simulink model "HRES_ORC_PEM"  (R2025b)
settings: Solver=ode23t  StartTime=0.0  StopTime=35000  MaxStep=1728  RelTol=1e-3
model workspace (MAT data in the model file):
  CND_L = 10
  CND_T0 = 333.15
  CND_d = 0.012
  CND_n = 20
  CND_p0 = 150000
  GAS_Tmax = 430
  GAS_dT = 20
  GAS_kb = 0.04
  GAS_ki = 0.002
  GAS_kp = 0.05
  GAS_min = 0.02
  GAS_total = 5
  GAS_u0 = 0.05
  HRS_L = 10
  HRS_LG = 1
  HRS_d = 0.012
  HRS_n = 6
  HRS_nG = 25
  HRS_p0 = 0.3
  HRS_x0 = 0.2
  NOZ_kb = 0.025
  NOZ_ki = 0.0005
  NOZ_kp = 0.02
  NOZ_min = 0.01
  NOZ_u0 = 0.1
  ORC_T3set = 400
  ORC_Taux = -2
  ORC_Taux0 = 0
  ORC_kb = 0.4
  ORC_ki = 2e-07
  ORC_kp = 5e-07
  ORC_mdot0 = 0.2
  ORC_mmax = 1
  ORC_mmin = 0.01
  ORC_pset_MPa = 1
  RCV_V = 0.2
  RCV_frac0 = 0.5
  RCV_p0 = 0.15
  RCV_tau = 0.1
  TRB_Tref = 400
  TRB_mdot = 0.6
  TRB_pr = 6
values from neighbouring files (symbols this model uses):
  R_h2 = 4.12    [run_simulation.m]
libraries: fl_lib x62, nesl_utility x56, SimscapeFluids_lib x9, slpidlib x4, ee_lib x2
(part 4 of 5)

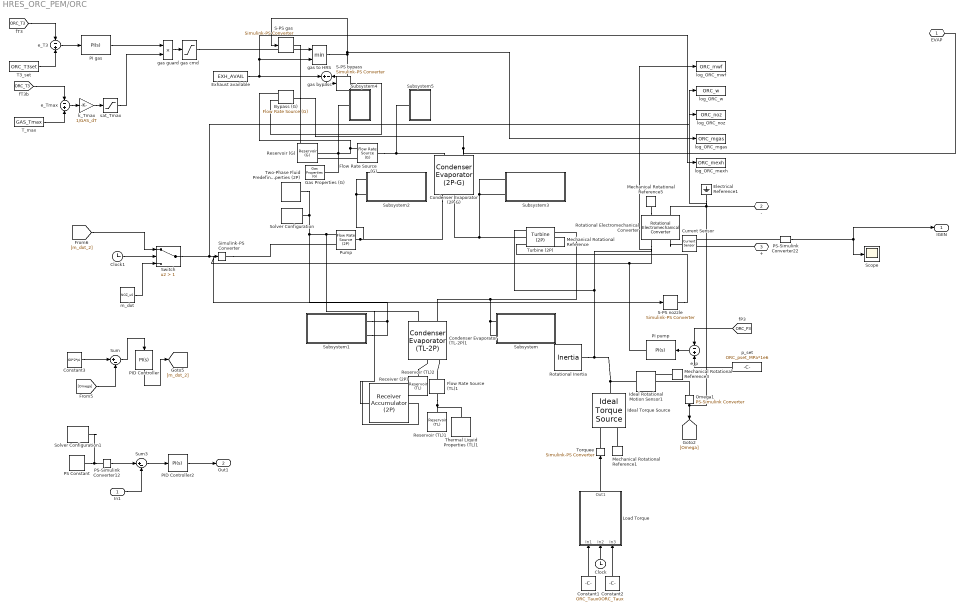
== system HRES_ORC_PEM/ORC ==
  In1 : Inport
  Bypass (G) : fl_lib/Gas/Sources/Flow Rate Source (G)  source_type=foundation.enum.constant_controlled.controlled  flow_type=foundation.enum.mass_volumetric_flow.mass  mass_flow=0 kg/s  volumetric_flow=0 m^3/s  volumetric_flow_conditions=foundation.enum.volumetric_flow_conditions.actual  p_std=0.101325 MPa  T_std=20 degC  power_spec=foundation.enum.power_spec.isentropic  area_A=0.01 m^2  area_B=0.01 m^2
      settings: InternalSimscapePortConfiguration="{\"Bottom\":[],\"Left\":[{\"id\":\"A\",\"label\":\"A\",\"type\":\"foundation.gas.gas\"},{\"id\":\"M\",\"label\":\"M\",\"type\":\"input\"}],\"Right\":[{\"id\":\"B\",\"label\":\"B\",\"type\":\"foundation.gas.gas\"}],\"Top\":[]}"
  Clock : Clock
  Clock1 : Clock
  Condenser Evaporator (2P-G) : SimscapeFluids_lib/Heat Exchangers/Two-Phase Fluid - Gas/Condenser Evaporator (2P-G)  flow_arrangement=fluids.heat_exchangers.enum.FlowArrangement2PG.Parallel  cross_flow_arrangement=fluids.heat_exchangers.enum.CrossFlowArrangement2PG.UnmixedUnmixed  R_wall=0 K/kW  wall_thermal_mass=false  mass_wall=1 kg  cp_wall=490 J/(K*kg)  area_A1=0.01 m^2  area_B1=0.01 m^2  area_A2=0.01 m^2  area_B2=0.01 m^2  tube_num_2P=HRS_n  tube_length_2P=HRS_L m  tube_cross_section_2P=fluids.heat_exchangers.enum.TubeCrossSection.Circular  tube_diameter_2P=HRS_d m  tube_width_2P=0.05 m  tube_height_2P=0.05 m  tube_inner_diameter_2P=0.05 m  tube_outer_diameter_2P=0.1 m  tube_flow_area_2P=0.002 m^2  tube_wetted_perimeter_2P=0.15 m  tube_heat_perimeter_2P=0.15 m  tube_pressure_loss_spec_2P=fluids.heat_exchangers.enum.TubePressureLossSpec2P.Haaland  tube_loss_coeff_2P=10  tube_local_pressure_loss_spec_2P=fluids.heat_exchangers.enum.LocalLossSpec.AggregateLength  tube_length_add_2P=0.1 m  tube_local_loss_coefficient_2P=0.1  tube_roughness_pressure_2P=15e-6 m  tube_Re_lam_pressure_2P=2000  tube_Re_tur_pressure_2P=4000  tube_shape_factor_generic_2P=64  tube_heat_coeff_spec_2P=fluids.heat_exchangers.enum.TubeHeatCoeffSpec2P.GneilinskiCavalliniZecchin  tube_colburn_coeff_liq_2P=[.023, .8, .33]  tube_colburn_coeff_mix_2P=[.05, .8, .33]  tube_colburn_coeff_vap_2P=[.023, .8, .33]  tube_roughness_heat_2P=15e-6 m  tube_Re_lam_heat_2P=2000  tube_Re_tur_heat_2P=4000  tube_Nu_lam_generic_2P=3.66  fouling_factor_2P=0.1 K*m^2/kW  fin_area_2P=0 m^2  fin_efficiency_2P=0.5  energy_spec_2P=foundation.enum.energy_spec.quality  p_init_2P=HRS_p0 MPa  T_init_2P=293.15 K  x_init_2P=HRS_x0  alpha_init_2P=0.5  h_init_2P=1500 kJ/kg  u_init_2P=1500 kJ/kg  flow_geometry_G=fluids.heat_exchangers.enum.FlowGeometryG.InsideTubes  tube_num_G=HRS_nG  tube_length_G=HRS_LG m  tube_cross_section_G=fluids.heat_exchangers.enum.TubeCrossSection.Circular  tube_diameter_G=0.05 m  tube_width_G=0.05 m  tube_height_G=0.05 m  tube_inner_diameter_G=0.05 m  tube_outer_diameter_G=0.1 m  tube_flow_area_G=0.002 m^2  tube_wetted_perimeter_G=0.15 m  tube_heat_perimeter_G=0.15 m  tube_pressure_loss_spec_G=fluids.heat_exchangers.enum.TubePressureLossSpec.Haaland  tube_loss_coeff_G=10  tube_local_pressure_loss_spec_G=fluids.heat_exchangers.enum.LocalLossSpec.AggregateLength  tube_length_add_G=0.1 m  tube_local_loss_coefficient_G=0.1  tube_roughness_pressure_G=15e-6 m  tube_Re_lam_pressure_G=2000  tube_Re_tur_pressure_G=4000  tube_shape_factor_generic_G=64  tube_heat_coeff_spec_G=fluids.heat_exchangers.enum.TubeHeatCoeffSpec.Gneilinski  tube_colburn_coeff_G=[.023, .8, .33]  tube_roughness_heat_G=15e-6 m  tube_Re_lam_heat_G=2000  tube_Re_tur_heat_G=4000  tube_Nu_lam_generic_G=3.66  bank_arrangement_G=fluids.heat_exchangers.enum.BankArrangement.Inline  bank_num_rows_G=5  bank_tubes_per_row_G=5  bank_width_G=1 m  bank_tube_diameter_G=0.05 m  bank_longitudinal_pitch_G=0.15 m  bank_transverse_pitch_G=0.15 m  bank_pressure_loss_spec_G=fluids.heat_exchangers.enum.BankPressureLossSpec.Martin  bank_euler_G=10  bank_heat_coeff_spec_G=fluids.heat_exchangers.enum.BankHeatCoeffSpec.Martin  bank_colburn_coeff_G=[.27, .63, .36]  generic_flow_area_G=0.01 m^2  generic_heat_area_G=2 m^2  generic_volume_G=0.05 m^3  generic_loss_coeff_G=10  generic_colburn_coeff_G=[.023, .8, .33]  fouling_factor_G=0.1 K*m^2/kW  fin_area_G=0 m^2  fin_efficiency_G=0.5  p_init_G=0.101325 MPa  T_init_G=453 K
      settings: InternalSimscapePortConfiguration="{\"Bottom\":[],\"Left\":[{\"id\":\"A1\",\"label\":\"A1\",\"type\":\"foundation.two_phase_fluid.two_phase_fluid\"},{\"id\":\"B1\",\"label\":\"B1\",\"type\":\"foundation.two_phase_fluid.two_phase_fluid\"}],\"Right\":[{\"id\":\"A2\",\"label\":\"A2\",\"type\":\"foundation.gas.gas\"},{\"id\":\"B2\",\"label\":\"B2\",\"type\":\"foundation.gas.gas\"}],\"Top\":[{\"id\":\"Z\",\"label\":\"Z\",\"type\":\"output\"}]}"
  Condenser Evaporator (TL-2P)1 : SimscapeFluids_lib/Heat Exchangers/Two-Phase Fluid - Thermal Liquid/Condenser Evaporator (TL-2P)  flow_arrangement=fluids.heat_exchangers.enum.FlowArrangementTL2P.Counter  cross_flow_arrangement=fluids.heat_exchangers.enum.CrossFlowArrangementTL2P.UnmixedUnmixed  R_wall=0 K/kW  wall_thermal_mass=false  mass_wall=1 kg  cp_wall=490 J/(K*kg)  area_A1=0.01 m^2  area_B1=0.01 m^2  area_A2=0.01 m^2  area_B2=0.01 m^2  flow_geometry_TL=fluids.heat_exchangers.enum.FlowGeometryTL.InsideTubes  tube_num_TL=40  tube_length_TL=1 m  tube_cross_section_TL=fluids.heat_exchangers.enum.TubeCrossSection.Circular  tube_diameter_TL=0.05 m  tube_width_TL=0.05 m  tube_height_TL=0.05 m  tube_inner_diameter_TL=0.05 m  tube_outer_diameter_TL=0.1 m  tube_flow_area_TL=0.002 m^2  tube_wetted_perimeter_TL=0.15 m  tube_heat_perimeter_TL=0.15 m  tube_pressure_loss_spec_TL=fluids.heat_exchangers.enum.TubePressureLossSpec.Haaland  tube_loss_coeff_TL=10  tube_local_pressure_loss_spec_TL=fluids.heat_exchangers.enum.LocalLossSpec.AggregateLength  tube_length_add_TL=0.1 m  tube_local_loss_coefficient_TL=0.1  tube_roughness_pressure_TL=15e-6 m  tube_Re_lam_pressure_TL=2000  tube_Re_tur_pressure_TL=4000  tube_shape_factor_generic_TL=64  tube_heat_coeff_spec_TL=fluids.heat_exchangers.enum.TubeHeatCoeffSpec.Gneilinski  tube_colburn_coeff_TL=[.023, .8, .33]  tube_roughness_heat_TL=15e-6 m  tube_Re_lam_heat_TL=2000  tube_Re_tur_heat_TL=4000  tube_Nu_lam_generic_TL=3.66  bank_arrangement_TL=fluids.heat_exchangers.enum.BankArrangement.Inline  bank_num_rows_TL=5  bank_tubes_per_row_TL=5  bank_width_TL=1 m  bank_tube_diameter_TL=0.05 m  bank_longitudinal_pitch_TL=0.15 m  bank_transverse_pitch_TL=0.15 m  bank_pressure_loss_spec_TL=fluids.heat_exchangers.enum.BankPressureLossSpec.Martin  bank_euler_TL=10  bank_heat_coeff_spec_TL=fluids.heat_exchangers.enum.BankHeatCoeffSpec.Martin  bank_colburn_coeff_TL=[.27, .63, .36]  generic_flow_area_TL=0.01 m^2  generic_heat_area_TL=2 m^2  generic_volume_TL=0.05 m^3  generic_loss_coeff_TL=10  generic_colburn_coeff_TL=[.023, .8, .33]  fouling_factor_TL=0.1 K*m^2/kW  fin_area_TL=0 m^2  fin_efficiency_TL=0.5  p_init_TL=99999 Pa  T_init_TL=275.15 K  tube_num_2P=CND_n  tube_length_2P=CND_L m  tube_cross_section_2P=fluids.heat_exchangers.enum.TubeCrossSection.Circular  tube_diameter_2P=CND_d m  tube_width_2P=0.05 m  tube_height_2P=0.05 m  tube_inner_diameter_2P=0.05 m  tube_outer_diameter_2P=0.1 m  tube_flow_area_2P=0.002 m^2  tube_wetted_perimeter_2P=0.15 m  tube_heat_perimeter_2P=0.15 m  tube_pressure_loss_spec_2P=fluids.heat_exchangers.enum.TubePressureLossSpec2P.Haaland  tube_loss_coeff_2P=10  tube_local_pressure_loss_spec_2P=fluids.heat_exchangers.enum.LocalLossSpec.AggregateLength  tube_length_add_2P=0.1 m  tube_local_loss_coefficient_2P=0.1  tube_roughness_pressure_2P=15e-6 m  tube_Re_lam_pressure_2P=2000  tube_Re_tur_pressure_2P=4000  tube_shape_factor_generic_2P=64  tube_heat_coeff_spec_2P=fluids.heat_exchangers.enum.TubeHeatCoeffSpec2P.GneilinskiCavalliniZecchin  tube_colburn_coeff_liq_2P=[.023, .8, .33]  tube_colburn_coeff_mix_2P=[.05, .8, .33]  tube_colburn_coeff_vap_2P=[.023, .8, .33]  tube_roughness_heat_2P=15e-6 m  tube_Re_lam_heat_2P=2000  tube_Re_tur_heat_2P=4000  tube_Nu_lam_generic_2P=3.66  fouling_factor_2P=0.1 K*m^2/kW  fin_area_2P=0 m^2  fin_efficiency_2P=0.5  energy_spec_2P=foundation.enum.energy_spec.temperature  p_init_2P=CND_p0 Pa  T_init_2P=CND_T0 K  x_init_2P=0.5  alpha_init_2P=0.5  h_init_2P=1500 kJ/kg  u_init_2P=1500 kJ/kg
      settings: InternalSimscapePortConfiguration="{\"Bottom\":[],\"Left\":[{\"id\":\"A1\",\"label\":\"A1\",\"type\":\"foundation.thermal_liquid.thermal_liquid\"},{\"id\":\"B1\",\"label\":\"B1\",\"type\":\"foundation.thermal_liquid.thermal_liquid\"}],\"Right\":[{\"id\":\"A2\",\"label\":\"A2\",\"type\":\"foundation.two_phase_fluid.two_phase_fluid\"},{\"id\":\"B2\",\"label\":\"B2\",\"type\":\"foundation.two_phase_fluid.two_phase_fluid\"}],\"Top\":[{\"id\":\"Z\",\"label\":\"Z\",\"type\":\"output\"}]}"
  Constant1 : Constant  Value=ORC_Taux0
  Constant2 : Constant  Value=ORC_Taux
  Constant3 : Constant  Value=60*2*pi
  Current Sensor : fl_lib/Electrical/Electrical Sensors/Current Sensor
  Electrical Reference1 : fl_lib/Electrical/Electrical Elements/Electrical Reference
  Exhaust available : FromWorkspace  VariableName=EXH_AVAIL  OutputAfterFinalValue=Holding final value
  Flow Rate Source (TL)1 : fl_lib/Thermal Liquid/Sources/Flow Rate Source (TL)  source_type=foundation.enum.constant_controlled.constant  flow_type=foundation.enum.mass_volumetric_flow.mass  mass_flow=15 kg/s  volumetric_flow=0 m^3/s  power_spec=foundation.enum.power_spec.isentropic  area=0.01 m^2
      settings: InternalSimscapePortConfiguration="{\"Bottom\":[],\"Left\":[{\"id\":\"A\",\"label\":\"A\",\"type\":\"foundation.thermal_liquid.thermal_liquid\"}],\"Right\":[{\"id\":\"B\",\"label\":\"B\",\"type\":\"foundation.thermal_liquid.thermal_liquid\"}],\"Top\":[]}"
  Flow Rate Source (G) : fl_lib/Gas/Sources/Flow Rate Source (G)  source_type=foundation.enum.constant_controlled.controlled  flow_type=foundation.enum.mass_volumetric_flow.mass  mass_flow=5 kg/s  volumetric_flow=0 m^3/s  volumetric_flow_conditions=foundation.enum.volumetric_flow_conditions.actual  p_std=0.101325 MPa  T_std=20 degC  power_spec=foundation.enum.power_spec.isentropic  area_A=0.01 m^2  area_B=0.01 m^2
      settings: InternalSimscapePortConfiguration="{\"Bottom\":[],\"Left\":[{\"id\":\"A\",\"label\":\"A\",\"type\":\"foundation.gas.gas\"},{\"id\":\"M\",\"label\":\"M\",\"type\":\"input\"}],\"Right\":[{\"id\":\"B\",\"label\":\"B\",\"type\":\"foundation.gas.gas\"}],\"Top\":[]}"
  Gas Properties (G) : fl_lib/Gas/Utilities/Gas Properties (G)  gas_spec=foundation.enum.gas_spec.perfect_gas  R=0.287 kJ/(K*kg)  Z=1  T_ref=293.15 K  h_ref=420 kJ/kg  cp_ref=1 kJ/(K*kg)  mu_ref=18 s*uPa  k_ref=26 mW/(K*m)  T_TLU1=[150 : 10 : 200, 250 : 50 : 1000, 1500, 2000]' K  h_TLU1=[275.264783730547; 285.377054177734; 295.474578903607; 305.560871069627; 315.638490783961; 325.709373787179; 376.008033649461; 426.297784741196; 476.678788323875; 527.253890684429; 578.12722735187; 629.395040865183; 681.137690131207; 733.415442873049; 786.267894376777; 839.715851152006; 893.764459999509; 948.406676876931; 1003.62653219711; 1059.40193232821; 1115.70691941005; 1172.51341226958; 1762.18512007361; 2377.14064127409] kJ/kg  cp_TLU1=[1.01211492398124; 1.01042105529234; 1.00914159006373; 1.00815898273273; 1.00739688341918; 1.00680484569075; 1.00554191216852; 1.00637389921747; 1.0092105862442; 1.01414404435034; 1.02111299587909; 1.02986878923959; 1.04003820504128; 1.05120320041448; 1.06296312852444; 1.07497111709439; 1.08694865668905; 1.0986858495625; 1.11003396604319; 1.12089493621399; 1.13121051694521; 1.14095251451866; 1.21001953144; 1.24628356718428] kJ/(K*kg)  mu_TLU1=[10.3766056544352; 10.9908682444892; 11.5932000841352; 12.1841060353213; 12.764067709023; 13.3335437107148; 16.038149065057; 18.5373404836509; 20.8671495114253; 23.0554226800681; 25.1239717991959; 27.0901379793485; 28.96790749834; 30.7687111230031; 32.5020036481173; 34.17569027566; 35.7964450415303; 37.3699520751368; 38.9010908824946; 40.3940804368247; 41.8525925389218; 43.279841956487; 56.3254722619962; 68.068290080945] s*uPa  k_TLU1=[14.1517155766309; 15.0474512994325; 15.9300520513026; 16.7998749295306; 17.6573089963228; 18.5027588910197; 22.5644026699512; 26.384465676638; 30.0032801168886; 33.4532006033488; 36.7600619429332; 39.9446251241844; 43.0237448740114; 46.0112537033799; 48.9186234516389; 51.7554617696538; 54.5298878921773; 57.2488200454925; 59.9181976996146; 62.5431553064749; 65.128159527924; 67.6771186900213; 91.7815514375552; 114.486299090693] mW/(K*m)  T_TLU2=[150 : 10 : 200, 250 : 50 : 1000, 1500, 2000]' K  p_TLU2=[0.001, 0.005, 0.01 : 0.01 : 0.1, 0.12, 0.15, 0.2, 0.5, 1, 2, 5, 10] MPa  rho_TLU2=[.0232262435294122, .116159536418799, .232389928446798, .465063671432694, .698022015548056, .931265751213184, 1.16479567270147, 1.39861257816015, 1.6327172696322, 1.86711055307826, 2.10179323839862, 2.33676613945539, 2.80758586416975, 3.5160126461103, 4.70263894299404, 11.983516436453, 24.7878864888476, 53.4753944012435, 188.202476404452, 488.088746553617; .0217743613495483, .108893511712, .217841319668304, .43590005028115, .654176644853253, .872671558133916, 1.09138524660849, 1.31031816850974, 1.52947078382145, 1.74884355428525, 1.96843694340691, 2.18825141646267, 2.62854548437173, 3.29065645015247, 4.39865940277095, 11.1676860192343, 22.9408518273177, 48.6188318442922, 151.41140977555, 397.086323615566; .0204933366521843, .102483510434793, .205009108095605, .410186693889784, .615533015460279, .821048331668635, 1.02673290215943, 1.23258698736378, 1.43861084849942, 1.64480474757224, 1.85116894737755, 2.05770371150129, 2.47128599100851, 3.09294527790581, 4.13249094693848, 10.4620818492884, 21.3797637857971, 44.7465382224065, 130.788260466556, 323.533424670971; .0193546817661166, .0967865758150396, .193606079729805, .38734394286521, .581213731637423, .775215588625983, .969349656759853, 1.16361607931376, 1.3580149999119, 1.55254656252557, 1.74721091147342, 1.94200819142115, 2.33200212471295, 2.91799364372034, 3.89732426996839, 9.84460606064557, 20.0372743829505, 41.551685035359, 116.744404785154, 273.404057887341; .0183359096145539, .0916899272240984, .183405807765996, .36691546510227, .55052904470126, .73424661940584, .918068262208759, 1.10199404625358, 1.28602404482977, 1.4701583313773, 1.65439697948324, 1.83874006288175, 2.20773983122517, 2.762024600182, 3.68793116346732, 9.2989642809239, 18.8669316601087, 38.8510263281099, 106.248040134752, 239.063674783047; .01741903255699, .0871033908068388, .174227353976232, .348537012803259, .52292900732162, .697403368434475, .871960127107058, 1.04659931436613, 1.22132096130094, 1.39612509905803, 1.57101175884641, 1.74598097193374, 2.09616718336943, 2.62206643530815, 3.50022045445381, 8.81280884432948, 17.8353318467781, 36.5262009931833, 97.9572133071041, 214.144269454883; .013935029468547, .069677797422131, .139362218300841, .278750918818379, .418166078341516, .557607673672086, .697075681624698, .836570079026588, .976090842717464, 1.11563794954935, 1.25521137638644, 1.39481110010495, 1.67408934575015, 2.09320336340731, 2.79224958681861, 7.00009934436889, 14.0635945083875, 28.3693859898697, 72.4958995959279, 148.061190553083; .0116124502542183, .0580629736195308, .116127751690325, .232262711724454, .348404861191252, .464554181197709, .580710652868886, .696874257347851, .813044975795622, .9292227893911, 1.04540767933102, 1.16159962682988, 1.3940046194509, 1.74266457145192, 2.32390314733333, 5.81485119489922, 11.6454651017326, 23.345179818482, 58.6036404676478, 116.933272564178; .0099534967844241, .0497674630503702, .0995348730218713, .199069527735142, .298603952162752, .39813813434232, .497672062326111, .597205724181, .696739107988446, .796272201844446, .89580499385952, .995337472158662, 1.19440144018133, 1.49299474329964, 1.99064239855983, 4.97624478331013, 9.95052507838832, 19.8877675359538, 49.5222664696343, 97.8281817865855; .00870929477376754, .0435461574066765, .0870915231079571, .174179875730153, .261265050544649, .348347040239765, .435425837514054, .522501435076285, .609573825645425, .696643001950612, .783708956731145, .870771682736456, 1.0448874194697, 1.30603662807179, 1.74121977223468, 4.35055112014231, 8.6923131825558, 17.3462098741118, 43.0204270425471, 84.5862815012905; .00774158811214905, .0387075144483394, .0774139632775453, .154823661826077, .232229091144957, .309630246740453, .387027124125729, .464419718820829, .541808026352667, .619192042255013, .696571762068483, .773947181340524, .92868510048419, 1.16075961421661, 1.54746386958083, 3.86538722275345, 7.71958432856407, 15.3924298760864, 38.0966874262009, 74.7409240194489; .00696742576213167, .0348366745541997, ...(+4677 chars)] kg/m^3  s_TLU2=[4.51795188269071, 4.05581817155212, 3.85666832168988, 3.65733557342939, 3.54058125651975, 3.45763599951791, 3.39321600973057, 3.34051347760226, 3.2958969095816, 3.25719862711102, 3.22302043260479, 3.19240764614444, 3.13933271586112, 3.07416650003008, 2.98972303348322, 2.71525667312277, 2.4961408855038, 2.25200576011077, 1.78471429674036, 1.29090458888978; 4.58264139768585, 4.12053027678858, 3.92140869957028, 3.72213261304626, 3.60543511368002, 3.52254683068083, 3.45818397201293, 3.40553872878098, 3.36097960809753, 3.32233893207258, 3.28821850379162, 3.25766364401107, 3.20470505116893, 3.13971456199421, 3.0555672742907, 2.78296953737326, 2.56736420779637, 2.33223141053168, 1.92951303779799, 1.47834112059833; 4.64340807746311, 4.18131468716962, 3.98221529565273, 3.7829836555054, 3.66633070274765, 3.58348706691023, 3.51916895627942, 3.46656856228366, 3.42205439236042, 3.38345876894588, 3.34938349545299, 3.31887389296688, 3.26600612355405, 3.20115264661303, 3.11723580728132, 2.84607806940339, 2.63311263769974, 2.40436393408814, 2.03542502560031, 1.64260706565665; 4.70070120514689, 4.23862199210925, 4.03954033696417, 3.84034421897669, 3.72372685440119, 3.64091887292993, 3.57663648301021, 3.52407187623307, 3.47959356019832, 3.44103385750504, 3.40699457172949, 3.37652102412054, 3.32372556659858, 3.25898106531012, 3.17524721731924, 2.90522439822934, 2.69430151549255, 2.47029333509785, 2.12268019468985, 1.77344207366055; 4.75489722787718, 4.29282953355363, 4.09376228675006, 3.89459501864723, 3.77800654829308, 3.6952275054615, 3.63097409868183, 3.57843851962613, 3.53398927597682, 3.49545869041481, 3.46144856659854, 3.43100422585914, 3.37826731713668, 3.31361097793741, 3.23002497599441, 2.96091365856363, 2.75160785927873, 2.5312406415135, 2.19841869007162, 1.87901583141216; 4.80631476306848, 4.34425655817633, 4.14520117995298, 3.94605767166668, 3.82949299137135, 3.74673776888186, 3.68250821276855, 3.6299965147449, 3.58557118253351, 3.54706453885701, 3.51307838741468, 3.48265804957869, 3.42996923841567, 3.36538527555295, 3.28192051690123, 3.0135531037355, 2.80555209686157, 2.58805540086205, 2.26610502263839, 1.96775904763196; 5.03005784939063, 4.56802897988245, 4.36901028390122, 4.16994018348893, 4.05344896894834, 3.97076727012748, 3.90661129562974, 3.85417323720152, 3.80982160259854, 3.77138871457567, 3.73747637686492, 3.70712991087092, 3.65458901785221, 3.59022736883767, 3.5071342997304, 3.24102784511277, 3.03691403727937, 2.82764560970477, 2.53381584725277, 2.28577338343632; 5.213071332015, 4.75105689184319, 4.55205623466113, 4.35302221894054, 4.23656709854542, 4.15392150331888, 4.08980164185938, 4.03739970590832, 3.99308420321641, 3.95468745653345, 3.92081126958634, 3.89050096377458, 3.83803241935538, 3.77377936374874, 3.69086747132005, 3.42585296452877, 3.22357730852106, 3.01804958620108, 2.73582153398541, 2.50683391368241; 5.36818677114197, 4.90618047542133, 4.70718999888292, 4.5081763447144, 4.391741586223, 4.30911635325018, 4.24501685439271, 4.19263528139031, 4.14834014199198, 4.10996375894582, 4.07610793597701, 4.04581799448331, 3.99339017971249, 3.92919822108258, 3.84638816350602, 3.58198482518679, 3.38072826636793, 3.17723930571407, 2.90109390657126, 2.68174878534546; 5.50312059773904, 5.04111933360368, 4.84213514624873, 4.64313406945348, 4.52671188701069, 4.444099228762, 4.38001230330443, 4.32764330237786, 4.28336073373153, 4.2449969201137, 4.21115366524977, 4.18087629053765, 4.12847360536087, 4.06431933120169, 3.98157205463241, 3.71754470888327, 3.51691216187067, 3.31466120289276, 3.04214220284213, 2.82845136827457; 5.62286980836317, 5.16087185851824, 4.96189181371153, 4.76289902096378, 4.64648512117041, 4.5638807441738, 4.49980209857165, 4.44744137610457, 4.40316708452248, 4.36481154657435, 4.33097656598627, 4.30070746415684, 4.24832132056873, 4.184191848361, 4.10148588060503, 3.83770566300567, 3.63748226836764, 3.43603958793625, 3.1658665252885, 2.9558053312017; 5.7308363809493, 5.26884072164272, 5.06986353974934, ...(+4595 chars)] kJ/(K*kg)  h_TLU2=[276.08088424589, 276.048494255671, 276.007989595737, 275.926922934925, 275.845779642901, 275.764559507019, 275.68326231383, 275.601887849085, 275.520435897725, 275.438906243879, 275.357298670861, 275.275612961165, 275.112006257597, 274.86600469197, 274.45440990197, 271.941510053176, 267.573991878308, 258.028969756929, 218.234362269026, 158.930370089034; 286.104280121225, 286.075386875978, 286.039258534729, 285.966962517021, 285.894613959392, 285.822212750054, 285.749758776967, 285.677251927836, 285.604692090115, 285.532079151003, 285.459412997448, 285.386693516142, 285.241094115775, 285.02229220976, 284.656540566853, 282.432853052032, 278.608576829258, 270.456137821523, 240.62825338508, 187.975341616082; 296.127712933609, 296.101741810155, 296.069269816893, 296.004298839236, 295.939291824284, 295.874248713054, 295.809169446516, 295.744053965591, 295.678902211156, 295.613714124043, 295.548489645037, 295.483228714877, 295.352597263841, 295.15637521962, 294.828601531559, 292.84221621424, 289.452931620771, 282.352183856267, 258.083267319111, 215.051052511419; 306.15128235, 306.127789707445, 306.098418400666, 306.03965742714, 305.980871947927, 305.922061932168, 305.863227349031, 305.804368167707, 305.745484357418, 305.686575887409, 305.627642726955, 305.568684845356, 305.450694796075, 305.273523547766, 304.977739633649, 303.189749788045, 300.157496456351, 293.885241012016, 273.341211471863, 237.921819553097; 316.175106263887, 316.153742662618, 316.127034494775, 316.073605930689, 316.02016104886, 315.966699833479, 315.913222268783, 315.859728339056, 315.806218028628, 315.752691321877, 315.69914820323, 315.64558865716, 315.538420220892, 315.377543975481, 315.109086307672, 313.489564435311, 310.756170955578, 305.156737704007, 287.344997830989, 257.435968836394; 326.199329972833, 326.179815330189, 326.155419682752, 326.106620570346, 326.057811027999, 326.008991047875, 325.960160622186, 325.911319743189, 325.862468403192, 325.813606594551, 325.764734309671, 325.715851541006, 325.61805452238, 325.471280180241, 325.226445621544, 323.751863790821, 321.272681065641, 316.232458831075, 300.538097964225, 274.729457520261; 376.334239729127, 376.321229547392, 376.304967312284, 376.272444481832, 376.239923836974, 376.207405376818, 376.174889100496, 376.142375007157, 376.109863095975, 376.077353366143, 376.044845816876, 376.012340447409, 375.94733624493, 375.849846271845, 375.687406489001, 374.713906995184, 373.095751316588, 369.876236784684, 360.387900683659, 345.656435942873; 426.525281394678, 426.516201936382, 426.50485367445, 426.482160685975, 426.459472409486, 426.436788842749, 426.414109983542, 426.391435829652, 426.36876637888, 426.346101629033, 426.323441577933, 426.30078622341, 426.255489595469, 426.18757982426, 426.074490520224, 425.398399641627, 424.280795394447, 422.079563123224, 415.746855514936, 406.194464895021; 476.840330742115, 476.833880716237, 476.825819267465, 476.80969998052, 476.793585505402, 476.777475839349, 476.761370979607, 476.745270923427, 476.729175668068, 476.713085210797, 476.696999548886, 476.680918679615, 476.648771308144, 476.600586128119, 476.520372988485, 476.041583484634, 475.252944483118, 473.709732112807, 469.339610018801, 462.897504479846; 527.36836576253, 527.363793291798, 527.358078674724, 527.346652677109, 527.335230992635, 527.323813618625, 527.312400552407, 527.300991791313, 527.289587332681, 527.278187173855, 527.26679131218, 527.255399745011, 527.232629483622, 527.198506234422, 527.141719692163, 526.803228763503, 526.247426409769, 525.16611881262, 522.148839900958, 517.815837109305; 578.206537117266, 578.203367844661, 578.199407091628, 578.191488376844, 578.183573381787, 578.175662104083, 578.16775454136, 578.159850691251, 578.151950551393, 578.144054119424, 578.136161392988, 578.128272369734, 578.112505423374, 578.088882719087, 578.049585297172, 577.815721490642, 577.433139940652, 576.694019389874, 574.669839072011, 571.873288825611; 629.447171720403, 629.445087134045, 629.442482115764, ...(+4600 chars)] kJ/kg  cp_TLU2=[1.00234082589656, 1.00272486727657, 1.00320557010184, 1.0041691525775, 1.00513564892549, 1.00610507294701, 1.00707743852905, 1.00805275964505, 1.00903105035552, 1.01001232480866, 1.01099659724104, 1.01198388197822, 1.01396754611819, 1.01696599794404, 1.02202562270308, 1.05412155485561, 1.1152747482059, 1.27776397304517, 2.72714600163742, 2.84169679152775; 1.00233987250094, 1.0026582461868, 1.00305665529268, 1.00385495020235, 1.00465521997313, 1.00545747174991, 1.00626171270995, 1.00706795006302, 1.00787619105157, 1.00868644295088, 1.00949871306922, 1.01031300874797, 1.01194770631902, 1.01441512983688, 1.01856901047877, 1.04463433942978, 1.09292211458076, 1.21254825029424, 1.91568051250176, 2.88130807863504; 1.00234833231511, 1.00261653513243, 1.00295209523415, 1.00362423915973, 1.00429775119299, 1.00497263511814, 1.00564889473126, 1.00632653384032, 1.00700555626519, 1.0076859658377, 1.00836776640166, 1.00905096181284, 1.01042155266012, 1.01248799737206, 1.01596048941702, 1.03756832264122, 1.07677086800609, 1.16935473257714, 1.61274080548658, 2.49705970753673; 1.00236750063458, 1.00259654480088, 1.00288306639866, 1.00345683185285, 1.00403156200318, 1.00460725887464, 1.00518392449607, 1.00576156090019, 1.00634017012356, 1.00691975420659, 1.00750031519354, 1.0080818551325, 1.00924788007791, 1.01100431105794, 1.013951550188, 1.03217016931395, 1.0646970984316, 1.13890069327182, 1.45314157485364, 2.09724000634052; 1.00239969156178, 1.00259759927889, 1.00284513880189, 1.00334073461589, 1.00383702035376, 1.00433399709602, 1.00483166592398, 1.00533002791975, 1.00582908416621, 1.00632883574697, 1.00682928374643, 1.00733042924969, 1.0083348171117, 1.00984665735215, 1.01238048621931, 1.02796073691597, 1.05542748615461, 1.11647221332449, 1.35460688567128, 1.82497183987797; 1.00244804156574, 1.00262078637436, 1.00283682944629, 1.00326928939605, 1.00370224822494, 1.00413570649822, 1.00456966478083, 1.00500412363741, 1.00543908363227, 1.00587454532937, 1.00631050929234, 1.00674697608445, 1.00762142040731, 1.0089368721703, 1.01113942325315, 1.02462437914299, 1.04815719159727, 1.09940879194009, 1.2879608304898, 1.64561032045572; 1.00307882131825, 1.00317682314491, 1.00329934910967, 1.00354447996773, 1.00378971604674, 1.0040350573259, 1.00428050378407, 1.0045260553997, 1.00477171215092, 1.00501747401546, 1.00526334097071, 1.00550931299369, 1.00600157214899, 1.00674074829383, 1.00797480662471, 1.01543403864644, 1.02807301255901, 1.05410032215668, 1.1370595668667, 1.27667353640799; 1.00479184412812, 1.00485489084091, 1.00493370280677, 1.00509133864519, 1.00524899034242, 1.00540665787824, 1.00556434123231, 1.00572204038417, 1.00587975531325, 1.00603748599888, 1.00619523242026, 1.00635299455648, 1.00666856588924, 1.00714204022039, 1.0079314755531, 1.01267611184663, 1.02061296964177, 1.03658189787277, 1.08483165641663, 1.16220451192724; 1.00811130709887, 1.00815514890263, 1.0082099496314, 1.00831954600127, 1.00842913558537, 1.008538718381, 1.0086482943854, 1.00875786359578, 1.00886742600928, 1.00897698162301, 1.00908653043401, 1.00919607243928, 1.00941513602039, 1.00974368027124, 1.01029111748123, 1.01357213131286, 1.01902645924599, 1.02987923459813, 1.06187268740862, 1.11203831447519; 1.01333843489686, 1.01337057745399, 1.01341075301128, 1.01349109533105, 1.01357142592839, 1.01365174480808, 1.01373205197484, 1.01381234743337, 1.01389263118834, 1.01397290324438, 1.01405316360612, 1.01413341227812, 1.01429387457109, 1.01453448045032, 1.01493525704896, 1.0173338224635, 1.02130841135621, 1.02917221070611, 1.05207076302405, 1.08759133887527; 1.0204993943148, 1.02052388121133, 1.02055448721779, 1.02061569051992, 1.02067688221331, 1.02073806230475, 1.02079923080097, 1.02086038770873, 1.02092153303472, 1.02098266678564, 1.02104378896817, 1.02110489958894, 1.02122708617172, 1.02141027949782, 1.02171537134855, 1.02353991759304, 1.02655828571218, 1.03251272842721, 1.04974356502866, 1.07634460433342; 1.02938754560642, 1.02940675254747, 1.02943075893538, ...(+4595 chars)] kJ/(K*kg)  mu_TLU2=[10.3589401268092, 10.3596215490306, 10.3604759816291, 10.3621937105615, 10.3639232830336, 10.3656647294411, 10.367418080323, 10.3691833663632, 10.3709606183908, 10.3727498673813, 10.3745511444581, 10.3763644808926, 10.3800274576703, 10.3856131584654, 10.3951680979376, 10.4591651061333, 10.5933716881858, 10.987254253246, 14.2772531553238, 32.0640438449792; 10.9730737505367, 10.9737639649823, 10.9746289690763, 10.9763664398934, 10.9781138770161, 10.9798712998652, 10.9816387279312, 10.9834161807751, 10.9852036780281, 10.9870012393928, 10.9888088846429, 10.9906266336238, 10.9942925225212, 10.9998676341554, 11.0093642467284, 11.0718587716065, 11.1983236137388, 11.5473941927686, 13.80253919041, 24.9939602435999; 11.5754207794231, 11.5761133162488, 11.5769808861739, 11.5787223615312, 11.5804722945392, 11.5822306975962, 11.583997583134, 11.5857729636177, 11.5875568515461, 11.5893492594517, 11.591150199901, 11.5929596854945, 11.5966043426875, 11.6021357340476, 11.6115273211419, 11.6724951531801, 11.7924961900945, 12.1087051696631, 13.877110798453, 21.116594552727; 12.1664431085071, 12.1671333783131, 12.1679978404446, 12.1697321846652, 12.1714737620145, 12.1732225803281, 12.1749786474567, 12.1767419712661, 12.1785125596373, 12.1802904204668, 12.1820755616661, 12.1838679911623, 12.1874747468313, 12.1929397416303, 12.2021948975387, 12.2616345418299, 12.3760758859915, 12.6668675990252, 14.1428657176503, 19.3071407602894; 12.7465920145367, 12.7472767611305, 12.7481340945151, 12.7498534307175, 12.7515789968564, 12.7533107977678, 12.7550488382933, 12.7567931232811, 12.7585436575851, 12.7603004460656, 12.7620634935889, 12.7638328050275, 12.7673902391718, 12.7727734919239, 12.7818715111764, 12.8397983982715, 12.9493527652261, 13.219710064689, 14.4977302956073, 18.4912497838941; 13.3163044188547, 13.3169813431509, 13.3178287127886, 13.3195275009732, 13.3212316900751, 13.3229412829416, 13.3246562824217, 13.3263766913661, 13.3281025126272, 13.3298337490592, 13.3315704035178, 13.3333124788606, 13.3368129036379, 13.3421042689754, 13.3510320108467, 13.4074736485989, 13.5126622664861, 13.7661027806947, 14.899955910071, 18.1598898734484; 16.0224075724356, 16.0230296694276, 16.0238079360955, 16.0253666205878, 16.0269281728135, 16.0284925922022, 16.0300598781818, 16.0316300301796, 16.0332030476219, 16.0347789299336, 16.0363576765389, 16.0379392868608, 16.0411110963421, 16.045890273958, 16.053912766856, 16.1035452030589, 16.191935922972, 16.3896878927643, 17.1441537726836, 18.884784635824; 18.5231398299684, 18.5237027673646, 18.52440681911, 18.5258161888637, 18.5272272462574, 18.5286399904383, 18.5300544205539, 18.5314705357511, 18.5328883351772, 18.534307817979, 18.5357289833034, 18.5371518302972, 18.5400025658792, 18.5442912604355, 18.5514726042656, 18.5954348735271, 18.6719871639656, 18.8370142902459, 19.4199345833489, 20.6372440527557; 20.8543235267059, 20.8548328470845, 20.8554697382748, 20.8567443227183, 20.8580199760048, 20.8592966974454, 20.8605744863513, 20.8618533420341, 20.8631332638056, 20.8644142509776, 20.8656963028623, 20.8669794187721, 20.8695488399177, 20.8734109346463, 20.8798689481311, 20.9191686895803, 20.986731360858, 21.1292934645023, 21.6108097810363, 22.5597942408407; 23.0437806943068, 23.0442434890065, 23.0448221434545, 23.045979989021, 23.0471385497258, 23.0482978250621, 23.0494578145236, 23.0506185176039, 23.0517799337972, 23.0529420625977, 23.0541049035001, 23.0552684559991, 23.0575976937678, 23.0610968747814, 23.066943007854, 23.1023882980934, 23.1628395000098, 23.2886837392316, 23.7017174154222, 24.4855712668615; 25.1133425341685, 25.1137653667077, 25.1142940198393, 25.1153517007868, 25.1164098810071, 25.1174685601327, 25.1185277377966, 25.1195874136318, 25.1206475872716, 25.1217082583496, 25.1227694264994, 25.1238310913551, 25.125955909721, 25.1291468534258, 25.134474978366, 25.1667008098841, 25.2213696262148, 25.3341476729655, 25.6971247787102, 26.3680691177854; 27.0803771465833, 27.0807656212508, 27.0812512958046, ...(+4595 chars)] s*uPa  k_TLU2=[14.0836394676256, 14.0862942007498, 14.0896194596466, 14.0962928994967, 14.102997040872, 14.1097320212018, 14.1164979631452, 14.1232949816993, 14.1301231872323, 14.1369826870758, 14.143873586467, 14.1507959891554, 14.1647357143434, 14.1858841226196, 14.2217750346856, 14.4546939871274, 14.9161812046845, 16.179147415959, 25.804405174674, 52.7180018225101; 14.9842167167395, 14.9866891286677, 14.9897852748967, 14.9959964117649, 15.002232761522, 15.0084944085447, 15.0147814269664, 15.021093885538, 15.0274318497018, 15.0337953826796, 15.0401845461169, 15.0465994004966, 15.0595064198135, 15.0790611017062, 15.1121738136527, 15.3249205125914, 15.7364707474682, 16.804366372496, 22.9562135535487, 43.3833329114209; 15.8710277123056, 15.8733403315285, 15.8762358183473, 15.8820425495945, 15.8878703464907, 15.8937192615434, 15.8995893400156, 15.9054806233308, 15.9113931505258, 15.9173269590121, 15.9232820850276, 15.9292585639261, 15.9412757184937, 15.9594624478981, 15.9902051816438, 16.1862002209989, 16.5586124847781, 17.4902098051164, 22.1528330719619, 36.7631825210105; 16.7445472483248, 16.7467187155221, 16.7494370491423, 16.7548870807582, 16.7603549672694, 16.765840741447, 16.7713444308513, 16.7768660602652, 16.7824056527314, 16.7879632300968, 16.7935388133348, 16.7991324227521, 16.8103737988234, 16.827371541412, 16.8560641436321, 17.0378636225901, 17.3785258158075, 18.208203678567, 22.0215304626411, 32.8930646908785; 17.6052538131622, 17.6072997236842, 17.6098605465768, 17.6149936632712, 17.6201420975008, 17.6253058695053, 17.630484995726, 17.6356794905705, 17.6408893671661, 17.6461146377541, 17.6513553139241, 17.6566114067637, 17.6671698848768, 17.6831234846882, 17.7100224746424, 17.8796016859028, 18.1938407516341, 18.9436656412164, 22.1982657206096, 30.777075291909; 18.4536214589847, 18.4555549890141, 18.4579748810943, 18.4628246117595, 18.4676876190316, 18.4725639150304, 18.4774535090791, 18.4823564089998, 18.4872726216651, 18.4922021532882, 18.4971450095944, 18.5021011959309, 18.5120535786224, 18.5270822466497, 18.5523972214712, 18.711323043571, 19.0031367814908, 19.6882500463792, 22.5419671243229, 29.6342111066617; 22.5261223969207, 22.5276347144758, 22.5295267397569, 22.5333162187732, 22.5371129348097, 22.5409168857571, 22.5447280689821, 22.5485464815665, 22.5523721204101, 22.5562049822839, 22.5600450638618, 22.5638923617408, 22.571608592487, 22.5832369726448, 22.6027614529468, 22.7236585032217, 22.9392024892054, 23.4208794883241, 25.2225807004481, 29.1026020666553; 26.3532131658036, 26.3544504957029, 26.3559981789686, 26.3590969468369, 26.36220024695, 26.3653080758599, 26.3684204301145, 26.3715373062584, 26.3746587008326, 26.3777846103743, 26.3809150314173, 26.3840499604917, 26.3903333288382, 26.3997921046468, 26.4156464271078, 26.513103457303, 26.6842088495029, 27.0572951588736, 28.3894828113755, 31.116172718458; 29.9769349622666, 29.9779792302173, 29.9792852821715, 29.9818997749358, 29.984517450741, 29.9871383070656, 29.9897623413869, 29.9923895511814, 29.9950199339243, 29.9976534870898, 30.000290208151, 30.00293009458, 30.0082193534245, 30.0161769186917, 30.0295024972172, 30.1110920118903, 30.2531619878245, 30.5589676635475, 31.6266997546166, 33.7713242983997; 33.4304742895722, 33.4313758571873, 33.4325033482028, 33.4347601010226, 33.4370192133728, 33.4392806834278, 33.4415445093619, 33.443810689349, 33.4460792215627, 33.4483501041766, 33.450623335364, 33.452898913298, 33.4574571020966, 33.464311940208, 33.4757833616242, 33.5458253676961, 33.6670810329056, 33.9257157838018, 34.8145797429682, 36.5779479385118; 36.7401102590657, 36.7409022384535, 36.7418926226882, 36.7438747571878, 36.7458587119437, 36.7478444856154, 36.7498320768626, 36.7518214843448, 36.7538127067217, 36.755805742653, 36.7578005907986, 36.7597972498181, 36.7637959951191, 36.7698076611259, 36.7798631433013, 36.8411331524036, 36.9467440951269, 37.1704725669481, 37.9301765555925, 39.4231380752276; 39.926865681602, 39.9275709717502, 39.9284529105416, ...(+4603 chars)] mW/(K*m)  beta_TLU2=[.000999939063271047, .00499847620325299, .00999390291790365, .019975596477506, .0299450577879351, .0399022638252297, .0498471914323395, .0597798173190184, .0697001180617656, .0796080701037593, .0895036497547952, .0993868331912267, .119115915458133, .148615963978671, .197531539031374, .484259268054388, .934728751330763, 1.71724988255064, 2.82175958388315, 17.9919018393343; .000999950175637603, .00499875419765594, .00999501582294484, .019980055533591, .0299551074444655, .039920159801454, .049875200783815, .0598202185046486, .069755201011013, .0796801362841905, .0895950122399321, .0994998167287049, .119279162382299, .148872337396356, .197991211869307, .487286155539529, .947989796271856, 1.78170846489774, 3.51015719198841, 10.7214594343083; .00099995895481445, .00499897378931246, .00999589475132194, .0199835757487714, .029963038080394, .0399342767982573, .049897286918626, .0598520634223456, .0697986012550663, .0797368953275347, .0896669405158784, .0995887316618911, .119407531024158, .149073693852866, .198351512022939, .489628938251755, .958019328446712, 1.82784028886759, 3.90652386037032, 8.82854192149657; .000999965991054188, .00499914976355599, .0099965989898174, .019986395438532, .0299693885486723, .0399455775011392, .0499149614555173, .0598775395501442, .0698333109025588, .0797822746096414, .0897244297478876, .0996597753736587, .11951003421407, .149234326410643, .198638486959409, .491476766853061, .965793651429376, 1.8622384486163, 4.16822627329493, 8.63159094055481; .000999971700637473, .00499929254433159, .00999717031901561, .0199886824058013, .0299745379437146, .0399547386012711, .0499292860323451, .0598981818764519, .0698614277587164, .0798190252903555, .0897709760687287, .0997172816775755, .119592963654789, .149364186682479, .198870192541928, .492957196986466, .971938886453558, 1.88865947552405, 4.35409769664694, 8.80496894225828; .000999976383827671, .00499940964837487, .00999763885669209, .0199905575293509, .029978759163036, .0399622468911828, .0499410238357645, .0599150931074531, .069884457805868, .0798491210194758, .0898090858260776, .09976435529279, .119660820422777, .149470379152736, .199059473751491, .494159033891154, .976874655018731, 1.90941822598397, 4.49230805929173, 9.03075785062252; .000999990490282384, .00499976233069882, .00999904969083958, .0199962017056947, .0299914604520388, .0399848303293515, .0499763157291795, .0599659210351961, .0699536506232617, .0799395088614837, .0899235001102771, .099905628722424, .119864315410104, .149788484054123, .199625422103725, .497712504275578, .991197318806328, 1.96746753165082, 4.84750864309542, 9.81988814731239; .000999996888689961, .00499992227353298, .00999968937543632, .0199987597506444, .0299972144943757, .0399950569692754, .0499922905319115, .0599889185328036, .0699849443164522, .0799803712213668, .0899752025800964, .0999694417192566, .119956156615841, .149931870141404, .199879988705673, .499290875622076, .99742780597502, 1.9917193153671, 4.98305568535804, 10.1656019796519; .00100000010404282, .00500000264124574, .0100000107657759, .0200000446683482, .0300001041122913, .0400001914978025, .0500003092207186, .0600004596725316, .0700006452404048, .0800008683071889, .0900011312514384, .100001436447427, .120002183070408, .150003679005398, .200007331564404, .500075036239648, 1.00048844086038, 2.0033761441506, 5.04492274361954, 10.3235244831897; .00100000181624883, .00500004543495486, .0100001818834321, .0200007286818531, .0300016421151244, .0400029239000145, .0500045757502084, .0600065993763173, .0700089964858884, .0800117687834143, .0900149179703425, .100018445745085, .120026643836544, .150041822669168, .200074917321734, .500489132153313, 1.00209119595608, 2.00937998338643, 5.07536569274062, 10.3970361107304; .00100000275171865, .00500006881389809, .0100002753602103, .0200011022772309, .0300024820039892, .0400044157912075, .0500069048874091, .0600099505389244, .070013553989897, .0800177164822894, .0900224392558898, .100027723548317, .120039981629321, .150062610958465, ...(+4923 chars)] MPa  alpha_TLU2=[.00666792026017809, .00667293852525301, .00667922012518017, .00669181264110188, .00670444439920956, .0067171155853866, .00672982638662978, .00674257699105705, .00675536758791526, .00676819836758812, .00678106952160409, .00679398124264439, .00681992716233515, .00685915517876874, .00692537286982025, .00734607851757868, .00815022150220267, .0102947700145685, .0286130234990625, .0187953609548895; .00625098287622453, .00625491678602209, .00625983959082828, .00626970330044927, .00627959121640412, .0062895034266007, .00629944001931492, .00630940108319236, .00631938670724969, .00632939698087609, .00633943199383484, .0063494918362647, .00636968637197943, .00640016667181258, .00645147598349833, .00677332847886827, .00736905474929384, .00884048760073163, .0171339202490674, .0215315077643186; .00588313555303659, .0058862675096628, .00589018585424886, .00589803389264854, .00590589709830074, .00591377551324048, .00592166917961251, .00592957813967143, .00593750243578164, .00594544211041737, .00595339720616273, .00596136776571166, .00597735544754535, .00600145402248875, .00604193334161856, .00629337413340494, .00674772192415558, .00781179743638987, .0126760057430892, .0188265238969795; .0055561870205014, .00555871383581219, .00556187450638498, .00556820302846878, .00557454114180011, .00558088886639395, .00558724622228694, .00559361322953698, .0055999899082232, .0056063762784456, .00561277236032489, .00561917817400221, .00563201907741633, .00565135392570052, .00568377600485627, .00588362426414759, .00623812701166661, .00703668964338148, .0102469955676518, .0149536825294414; .00526367328574603, .00526573545598588, .00526831453344121, .00527347724162598, .0052786460285981, .00528382090365857, .00528900187610229, .00529418895521789, .00529938215028738, .00530458147058612, .00530978692538254, .00531499852393791, .00532544018933368, .00534114899671789, .00536745444819242, .00552860555277807, .00581033085505093, .00642649496887873, .00869646281395399, .012066880795797; .00500042488960082, .00500212483016686, .00500425061604882, .00500850505700949, .00501276332697717, .00501702543003454, .0050212913702516, .00502556115168559, .00502983477838086, .0050341122543686, .00503839358366686, .00504267877028035, .00505126073140412, .00506416270228762, .00508574365995129, .00521729340118635, .00544459697246268, .00593041440285951, .0076105627631654, .0100682280023522; .00400018129970419, .00400090650861602, .00400181304245358, .00400362618568443, .00400543942947194, .00400725277359113, .00400906621781262, .00401087976190256, .00401269340562272, .00401450714873037, .00401632099097834, .00401813493211499, .00402176311002518, .00402720611200514, .00403627972376539, .00409077021034855, .00418174921054286, .00436400960219121, .00490100541701872, .00562155604159635; .00333342119928242, .00333377263203594, .00333421185313783, .00333509006258143, .00333596796174708, .0033368455507164, .00333772282956964, .0033385997983857, .00333947645724213, .00334035280621511, .00334122884537947, .00334210457480867, .00334385510474869, .00334647857840336, .00335084484885457, .00337688044325411, .00341965705023207, .00350288036408, .00373210009503289, .0040224471305652; .00285718871724807, .00285737213017767, .00285760133449809, .00285805953708679, .0028585174650906, .00285897511869055, .002859432498067, .00285988960339967, .00286034643486761, .00286080299264927, .00286125927692239, .00286171528786412, .00286262649045861, .00286399124875565, .0028662604025581, .00287973354731443, .00290165734133489, .00294356774142556, .00305431746464114, .00318740088788344; .00250002489125244, .00250012443655583, .00250024882385804, .00250049745078393, .00250074588094204, .00250099411449637, .00250124215161053, .00250148999244774, .00250173763717087, .00250198508594236, .00250223233892431, .00250247939627841, .002502972924748, .00250371175426422, .00250493924559049, .0025122030852077, .00252393267225762, .00254603777605415, .00260236336428197, .0026655593424356; .00222223585417192, ...(+5604 chars)/K  T_min_perfect=1 K  T_max_perfect=inf K  p_min_perfect=1 Pa  p_max_perfect=inf MPa  T_range_flag=foundation.enum.T_range_G.from_props  T_min_semiperfect=150 K  T_max_semiperfect=2000 K  p_min_semiperfect=1 Pa  p_max_semiperfect=inf MPa  pT_region_flag=foundation.enum.pT_region_G.from_props  pT_validity_TLU2=ones(24, 20)  T_min_real=150 K  T_max_real=2000 K  p_min_real=0.001 MPa  p_max_real=10 MPa  p_atm=0.101325 MPa  properties_range_check=simscape.enum.assert.action.error  Mach_rev=0.001
  Ideal Rotational Motion Sensor1 : fl_lib/Mechanical/Mechanical Sensors/Ideal Rotational Motion Sensor  reference=foundation.enum.MeasurementReference.difference  acceleration_port=false  velocity_port=true  position_port=true  wrap_angle=false  offset=0 rad
  Ideal Torque Source : fl_lib/Mechanical/Mechanical Sources/Ideal Torque Source
  Load Torque : Subsystem
  Mechanical Rotational Reference{,1,3,5} (4 alike) : fl_lib/Mechanical/Rotational Elements/Mechanical Rotational Reference
  Omega1 : nesl_utility/PS-Simulink Converter  PhysicalDomain=network_engine_domain  SubClassName=ps_output  LeftPortType=input  RightPortType=output  PseudoPeriodic=off  Frequencies=[]  VectorFormat=inherit  Unit=inherit  AffineConversion=off
  PI gas : slpidlib/PID Controller  Controller=PI  Form=Parallel  TimeDomain=Continuous-time  UseExternalTs=off  SampleTime=-1  IntegratorMethod=Forward Euler  FilterMethod=Forward Euler  ControllerParametersSource=internal  P=GAS_kp  I=GAS_ki  UseKiTs=off  D=0  UseExternalDerivativeSource=off  N=100  UseFilter=on  TunerSelectOption=Transfer Function Based (PID Tuner App)  ZeroCross=off  InitialConditionSource=internal  InitialConditionForIntegrator=GAS_u0  InitialConditionForFilter=0  DifferentiatorICPrevScaledInput=0  ExternalReset=none  TrackingMode=off  Kt=1  LimitOutput=on  SatLimitsSource=internal  UpperSaturationLimit=GAS_total  LowerSaturationLimit=GAS_min  LinearizeAsGain=on  AntiWindupMode=clamping  Kb=GAS_kb  LimitIntegrator=off  UpperIntegratorSaturationLimit=inf  LowerIntegratorSaturationLimit=-inf  POutMin=[]  POutMax=[]  IOutMin=[]  IOutMax=[]  DOutMin=[]  DOutMax=[]  NOutMin=[]  NOutMax=[]  SumOutMin=[]  SumOutMax=[]  SaturationOutMin=[]  SaturationOutMax=[]  PParamMin=[]  PParamMax=[]  IParamMin=[]  IParamMax=[]  DParamMin=[]  DParamMax=[]  NParamMin=[]  NParamMax=[]  KbParamMin=[]  KbParamMax=[]  KtParamMin=[]  KtParamMax=[]  KbOutMin=[]  KbOutMax=[]  KtOutMin=[]  KtOutMax=[]  IntegratorOutMin=[]  IntegratorOutMax=[]  FilterOutMin=[]  FilterOutMax=[]  SumI1OutMin=[]  SumI1OutMax=[]  SumI2OutMin=[]  SumI2OutMax=[]  SumI3OutMin=[]  SumI3OutMax=[]  SumI4OutMin=[]  SumI4OutMax=[]  SumDOutMin=[]  SumDOutMax=[]  DifferentiatorOutMin=[]  DifferentiatorOutMax=[]  FilterDiffOutCoefMin=[]  FilterDiffOutCoefMax=[]  ReciprocalOutMin=[]  ReciprocalOutMax=[]  SumDenOutMin=[]  SumDenOutMax=[]  SumNumOutMin=[]  SumNumOutMax=[]  DivideOutMin=[]  DivideOutMax=[]  UdiffTsProdOutMin=[]  UdiffTsProdOutMax=[]  NTsProdOutMin=[]  NTsProdOutMax=[]  UintegralTsProdOutMin=[]  UintegralTsProdOutMax=[]  UngainTsProdOutMin=[]  UngainTsProdOutMax=[]  ClampingZeroOutDataTypeStr=Inherit: Inherit via back propagation  ClampingZeroOutMin=[]  ClampingZeroOutMax=[]  FilterDenConstantOutDataTypeStr=Inherit: Inherit via back propagation  FilterDenConstantOutMin=[]  FilterDenConstantOutMax=[]  PCopyOutDataTypeStr=Inherit: Inherit via back propagation  PCopyOutMin=[]  PCopyOutMax=[]  NCopyOutDataTypeStr=Inherit: Inherit via back propagation  NCopyOutMin=[]  NCopyOutMax=[]  IntegratorContinuousStateAttributes=''  IntegratorStateMustResolveToSignalObject=off  IntegratorRTWStateStorageClass=Auto  FilterContinuousStateAttributes=''  FilterStateMustResolveToSignalObject=off  FilterRTWStateStorageClass=Auto  ParallelPVariant=InternalParameters  IdealPVariant=Disabled  IVariant=InternalParameters  DVariant=Disabled  IntegratorVariant=Continuous  SatVariant=Enabled  AWVariant=ContClampingParallel  PCopyVariant=Disabled  TRVariant=Disabled  FdbkBlocksVariant=Forward  IdealPFdbkVariant=Disabled  SatFdbkVariant=Disabled  DerivativeFilterVariant=Disabled  NVariant=Disabled  NCopyVariant=Disabled_SignalSpec  FilterICVariant=Disabled  IntegratorICVariant=InternalICs  ExternalResetVariant=Disabled  TRSumVariant=Passthrough  SumFdbkVariant=Disabled  SumVariant=Sum_PI  TsampFilterVariant=InternalTs  TsampNgainVariant=Passthrough  TsampIntegralVariant=Disabled_SignalSpec  ExternalSaturationOutDataTypeStr=Inherit: Same as second input  DerivativeSourceVariant=Disabled  PreIntVariant=InternalPreInt
  PI pump : slpidlib/PID Controller  Controller=PI  Form=Parallel  TimeDomain=Continuous-time  UseExternalTs=off  SampleTime=-1  IntegratorMethod=Forward Euler  FilterMethod=Forward Euler  ControllerParametersSource=internal  P=ORC_kp  I=ORC_ki  UseKiTs=off  D=0  UseExternalDerivativeSource=off  N=100  UseFilter=on  TunerSelectOption=Transfer Function Based (PID Tuner App)  ZeroCross=off  InitialConditionSource=internal  InitialConditionForIntegrator=ORC_mdot0  InitialConditionForFilter=0  DifferentiatorICPrevScaledInput=0  ExternalReset=none  TrackingMode=off  Kt=1  LimitOutput=on  SatLimitsSource=internal  UpperSaturationLimit=ORC_mmax  LowerSaturationLimit=ORC_mmin  LinearizeAsGain=on  AntiWindupMode=back-calculation  Kb=ORC_kb  LimitIntegrator=off  UpperIntegratorSaturationLimit=inf  LowerIntegratorSaturationLimit=-inf  POutMin=[]  POutMax=[]  IOutMin=[]  IOutMax=[]  DOutMin=[]  DOutMax=[]  NOutMin=[]  NOutMax=[]  SumOutMin=[]  SumOutMax=[]  SaturationOutMin=[]  SaturationOutMax=[]  PParamMin=[]  PParamMax=[]  IParamMin=[]  IParamMax=[]  DParamMin=[]  DParamMax=[]  NParamMin=[]  NParamMax=[]  KbParamMin=[]  KbParamMax=[]  KtParamMin=[]  KtParamMax=[]  KbOutMin=[]  KbOutMax=[]  KtOutMin=[]  KtOutMax=[]  IntegratorOutMin=[]  IntegratorOutMax=[]  FilterOutMin=[]  FilterOutMax=[]  SumI1OutMin=[]  SumI1OutMax=[]  SumI2OutMin=[]  SumI2OutMax=[]  SumI3OutMin=[]  SumI3OutMax=[]  SumI4OutMin=[]  SumI4OutMax=[]  SumDOutMin=[]  SumDOutMax=[]  DifferentiatorOutMin=[]  DifferentiatorOutMax=[]  FilterDiffOutCoefMin=[]  FilterDiffOutCoefMax=[]  ReciprocalOutMin=[]  ReciprocalOutMax=[]  SumDenOutMin=[]  SumDenOutMax=[]  SumNumOutMin=[]  SumNumOutMax=[]  DivideOutMin=[]  DivideOutMax=[]  UdiffTsProdOutMin=[]  UdiffTsProdOutMax=[]  NTsProdOutMin=[]  NTsProdOutMax=[]  UintegralTsProdOutMin=[]  UintegralTsProdOutMax=[]  UngainTsProdOutMin=[]  UngainTsProdOutMax=[]  ClampingZeroOutDataTypeStr=Inherit: Inherit via back propagation  ClampingZeroOutMin=[]  ClampingZeroOutMax=[]  FilterDenConstantOutDataTypeStr=Inherit: Inherit via back propagation  FilterDenConstantOutMin=[]  FilterDenConstantOutMax=[]  PCopyOutDataTypeStr=Inherit: Inherit via back propagation  PCopyOutMin=[]  PCopyOutMax=[]  NCopyOutDataTypeStr=Inherit: Inherit via back propagation  NCopyOutMin=[]  NCopyOutMax=[]  IntegratorContinuousStateAttributes=''  IntegratorStateMustResolveToSignalObject=off  IntegratorRTWStateStorageClass=Auto  FilterContinuousStateAttributes=''  FilterStateMustResolveToSignalObject=off  FilterRTWStateStorageClass=Auto  ParallelPVariant=InternalParameters  IdealPVariant=Disabled  IVariant=InternalParameters  DVariant=Disabled  IntegratorVariant=Continuous  SatVariant=Enabled  AWVariant=BackCalculation  PCopyVariant=Disabled  TRVariant=Disabled  FdbkBlocksVariant=Forward  IdealPFdbkVariant=Disabled  SatFdbkVariant=Disabled  DerivativeFilterVariant=Disabled  NVariant=Disabled  NCopyVariant=Disabled_SignalSpec  FilterICVariant=Disabled  IntegratorICVariant=InternalICs  ExternalResetVariant=Disabled  TRSumVariant=Passthrough  SumFdbkVariant=Disabled  SumVariant=Sum_PI  TsampFilterVariant=InternalTs  TsampNgainVariant=Passthrough  TsampIntegralVariant=Disabled_SignalSpec  ExternalSaturationOutDataTypeStr=Inherit: Same as second input  DerivativeSourceVariant=Disabled  PreIntVariant=InternalPreInt
  PID Controller : slpidlib/PID Controller  Controller=PI  Form=Parallel  TimeDomain=Continuous-time  UseExternalTs=off  SampleTime=-1  IntegratorMethod=Forward Euler  FilterMethod=Forward Euler  ControllerParametersSource=internal  P=NOZ_kp  I=NOZ_ki  UseKiTs=off  D=0  UseExternalDerivativeSource=off  N=100  UseFilter=on  TunerSelectOption=Transfer Function Based (PID Tuner App)  ZeroCross=off  InitialConditionSource=internal  InitialConditionForIntegrator=NOZ_u0  InitialConditionForFilter=0  DifferentiatorICPrevScaledInput=0  ExternalReset=none  TrackingMode=off  Kt=1  LimitOutput=on  SatLimitsSource=internal  UpperSaturationLimit=1  LowerSaturationLimit=NOZ_min  LinearizeAsGain=on  AntiWindupMode=clamping  Kb=NOZ_kb  LimitIntegrator=off  UpperIntegratorSaturationLimit=inf  LowerIntegratorSaturationLimit=-inf  POutMin=[]  POutMax=[]  IOutMin=[]  IOutMax=[]  DOutMin=[]  DOutMax=[]  NOutMin=[]  NOutMax=[]  SumOutMin=[]  SumOutMax=[]  SaturationOutMin=[]  SaturationOutMax=[]  PParamMin=[]  PParamMax=[]  IParamMin=[]  IParamMax=[]  DParamMin=[]  DParamMax=[]  NParamMin=[]  NParamMax=[]  KbParamMin=[]  KbParamMax=[]  KtParamMin=[]  KtParamMax=[]  KbOutMin=[]  KbOutMax=[]  KtOutMin=[]  KtOutMax=[]  IntegratorOutMin=[]  IntegratorOutMax=[]  FilterOutMin=[]  FilterOutMax=[]  SumI1OutMin=[]  SumI1OutMax=[]  SumI2OutMin=[]  SumI2OutMax=[]  SumI3OutMin=[]  SumI3OutMax=[]  SumI4OutMin=[]  SumI4OutMax=[]  SumDOutMin=[]  SumDOutMax=[]  DifferentiatorOutMin=[]  DifferentiatorOutMax=[]  FilterDiffOutCoefMin=[]  FilterDiffOutCoefMax=[]  ReciprocalOutMin=[]  ReciprocalOutMax=[]  SumDenOutMin=[]  SumDenOutMax=[]  SumNumOutMin=[]  SumNumOutMax=[]  DivideOutMin=[]  DivideOutMax=[]  UdiffTsProdOutMin=[]  UdiffTsProdOutMax=[]  NTsProdOutMin=[]  NTsProdOutMax=[]  UintegralTsProdOutMin=[]  UintegralTsProdOutMax=[]  UngainTsProdOutMin=[]  UngainTsProdOutMax=[]  ClampingZeroOutDataTypeStr=Inherit: Inherit via back propagation  ClampingZeroOutMin=[]  ClampingZeroOutMax=[]  FilterDenConstantOutDataTypeStr=Inherit: Inherit via back propagation  FilterDenConstantOutMin=[]  FilterDenConstantOutMax=[]  PCopyOutDataTypeStr=Inherit: Inherit via back propagation  PCopyOutMin=[]  PCopyOutMax=[]  NCopyOutDataTypeStr=Inherit: Inherit via back propagation  NCopyOutMin=[]  NCopyOutMax=[]  IntegratorContinuousStateAttributes=''  IntegratorStateMustResolveToSignalObject=off  IntegratorRTWStateStorageClass=Auto  FilterContinuousStateAttributes=''  FilterStateMustResolveToSignalObject=off  FilterRTWStateStorageClass=Auto  ParallelPVariant=InternalParameters  IdealPVariant=Disabled  IVariant=InternalParameters  DVariant=Disabled  IntegratorVariant=Continuous  SatVariant=Enabled  AWVariant=ContClampingParallel  PCopyVariant=Disabled  TRVariant=Disabled  FdbkBlocksVariant=Forward  IdealPFdbkVariant=Disabled  SatFdbkVariant=Disabled  DerivativeFilterVariant=Disabled  NVariant=Disabled  NCopyVariant=Disabled_SignalSpec  FilterICVariant=Disabled  IntegratorICVariant=InternalICs  ExternalResetVariant=Disabled  TRSumVariant=Passthrough  SumFdbkVariant=Disabled  SumVariant=Sum_PI  TsampFilterVariant=InternalTs  TsampNgainVariant=Passthrough  TsampIntegralVariant=Disabled_SignalSpec  ExternalSaturationOutDataTypeStr=Inherit: Same as second input  DerivativeSourceVariant=Disabled  PreIntVariant=InternalPreInt
  PID Controller2 : slpidlib/PID Controller  Controller=PI  Form=Parallel  TimeDomain=Continuous-time  UseExternalTs=off  SampleTime=-1  IntegratorMethod=Forward Euler  FilterMethod=Forward Euler  ControllerParametersSource=internal  P=80  I=8  UseKiTs=off  D=0  UseExternalDerivativeSource=off  N=100  UseFilter=on  TunerSelectOption=Transfer Function Based (PID Tuner App)  InitialConditionSource=internal  InitialConditionForIntegrator=0  InitialConditionForFilter=0  DifferentiatorICPrevScaledInput=0  ExternalReset=none  TrackingMode=off  Kt=1  LimitOutput=on  SatLimitsSource=internal  UpperSaturationLimit=1080  LowerSaturationLimit=0  LinearizeAsGain=on  AntiWindupMode=back-calculation  Kb=1  LimitIntegrator=off  UpperIntegratorSaturationLimit=inf  LowerIntegratorSaturationLimit=-inf  POutMin=[]  POutMax=[]  IOutMin=[]  IOutMax=[]  DOutMin=[]  DOutMax=[]  NOutMin=[]  NOutMax=[]  SumOutMin=[]  SumOutMax=[]  SaturationOutMin=[]  SaturationOutMax=[]  PParamMin=[]  PParamMax=[]  IParamMin=[]  IParamMax=[]  DParamMin=[]  DParamMax=[]  NParamMin=[]  NParamMax=[]  KbParamMin=[]  KbParamMax=[]  KtParamMin=[]  KtParamMax=[]  KbOutMin=[]  KbOutMax=[]  KtOutMin=[]  KtOutMax=[]  IntegratorOutMin=[]  IntegratorOutMax=[]  FilterOutMin=[]  FilterOutMax=[]  SumI1OutMin=[]  SumI1OutMax=[]  SumI2OutMin=[]  SumI2OutMax=[]  SumI3OutMin=[]  SumI3OutMax=[]  SumI4OutMin=[]  SumI4OutMax=[]  SumDOutMin=[]  SumDOutMax=[]  DifferentiatorOutMin=[]  DifferentiatorOutMax=[]  FilterDiffOutCoefMin=[]  FilterDiffOutCoefMax=[]  ReciprocalOutMin=[]  ReciprocalOutMax=[]  SumDenOutMin=[]  SumDenOutMax=[]  SumNumOutMin=[]  SumNumOutMax=[]  DivideOutMin=[]  DivideOutMax=[]  UdiffTsProdOutMin=[]  UdiffTsProdOutMax=[]  NTsProdOutMin=[]  NTsProdOutMax=[]  UintegralTsProdOutMin=[]  UintegralTsProdOutMax=[]  UngainTsProdOutMin=[]  UngainTsProdOutMax=[]  ClampingZeroOutDataTypeStr=Inherit: Inherit via back propagation  ClampingZeroOutMin=[]  ClampingZeroOutMax=[]  FilterDenConstantOutDataTypeStr=Inherit: Inherit via back propagation  FilterDenConstantOutMin=[]  FilterDenConstantOutMax=[]  PCopyOutDataTypeStr=Inherit: Inherit via back propagation  PCopyOutMin=[]  PCopyOutMax=[]  NCopyOutDataTypeStr=Inherit: Inherit via back propagation  NCopyOutMin=[]  NCopyOutMax=[]  IntegratorContinuousStateAttributes=''  IntegratorStateMustResolveToSignalObject=off  IntegratorRTWStateStorageClass=Auto  FilterContinuousStateAttributes=''  FilterStateMustResolveToSignalObject=off  FilterRTWStateStorageClass=Auto  ParallelPVariant=InternalParameters  IdealPVariant=Disabled  IVariant=InternalParameters  DVariant=Disabled  IntegratorVariant=Continuous  SatVariant=Enabled  AWVariant=BackCalculation  PCopyVariant=Disabled  TRVariant=Disabled  FdbkBlocksVariant=Forward  IdealPFdbkVariant=Disabled  SatFdbkVariant=Disabled  DerivativeFilterVariant=Disabled  NVariant=Disabled  NCopyVariant=Disabled_SignalSpec  FilterICVariant=Disabled  IntegratorICVariant=InternalICs  ExternalResetVariant=Disabled  TRSumVariant=Passthrough  SumFdbkVariant=Disabled  SumVariant=Sum_PI  TsampFilterVariant=InternalTs  TsampNgainVariant=Passthrough  TsampIntegralVariant=Disabled_SignalSpec  ExternalSaturationOutDataTypeStr=Inherit: Same as second input  DerivativeSourceVariant=Disabled  PreIntVariant=InternalPreInt
  PS Constant : fl_lib/Physical Signals/Sources/PS Constant  constant=360 K
  PS-Simulink Converter12 : nesl_utility/PS-Simulink Converter  PhysicalDomain=network_engine_domain  SubClassName=ps_output  LeftPortType=input  RightPortType=output  PseudoPeriodic=off  Frequencies=[]  VectorFormat=inherit  Unit=K  AffineConversion=off
  PS-Simulink Converter22 : nesl_utility/PS-Simulink Converter  PhysicalDomain=network_engine_domain  SubClassName=ps_output  LeftPortType=input  RightPortType=output  PseudoPeriodic=off  Frequencies=[]  VectorFormat=inherit  Unit=inherit  AffineConversion=off
  Pump : fl_lib/Two-Phase Fluid/Sources/Flow Rate Source (2P)  source_type=foundation.enum.constant_controlled.controlled  flow_type=foundation.enum.mass_volumetric_flow.mass  mass_flow=0.8 kg/s  volumetric_flow=0 m^3/s  power_spec=foundation.enum.power_spec.isentropic  area_A=0.01 m^2  area_B=0.01 m^2
      settings: InternalSimscapePortConfiguration="{\"Bottom\":[],\"Left\":[{\"id\":\"A\",\"label\":\"A\",\"type\":\"foundation.two_phase_fluid.two_phase_fluid\"},{\"id\":\"M\",\"label\":\"M\",\"type\":\"input\"}],\"Right\":[{\"id\":\"B\",\"label\":\"B\",\"type\":\"foundation.two_phase_fluid.two_phase_fluid\"}],\"Top\":[]}"
  Receiver (2P) : SimscapeFluids_lib/Two-Phase Fluid/Tanks & Accumulators/Receiver Accumulator (2P)  volume=RCV_V m^3  tank_area=0.5 m^2  area_AV=0.01 m^2  area_BV=0.01 m^2  area_AL=0.01 m^2  area_BL=0.01 m^2  V_frac_liq_error=simscape.enum.assert.action.none  V_frac_liq_min=0.05  V_frac_liq_max=0.95  V_frac_smooth=0.05  p_crit_error=simscape.enum.assert.action.error  hc_vap=20 W/(K*m^2)  hc_liq=100 W/(K*m^2)  p_init=RCV_p0 MPa  fraction_spec=fluids.two_phase_fluid.tanks_accumulators.enum.LiquidFractionSpec.Volume  M_frac_liq_init=0.5  V_frac_liq_init=RCV_frac0  saturated_init=true  energy_spec=fluids.two_phase_fluid.tanks_accumulators.enum.EnergySpec.SubcoolingSuperheating  delta_T_sub_init=5 deltaK  delta_T_sup_init=5 deltaK  T_liq_init=368.15 K  T_vap_init=378.15 K  h_liq_init=400 kJ/kg  h_vap_init=2700 kJ/kg  u_liq_init=400 kJ/kg  u_vap_init=2700 kJ/kg  tau_vap_cond=RCV_tau s
      settings: InternalSimscapePortConfiguration="{\"Bottom\":[],\"Left\":[{\"id\":\"AV\",\"label\":\"AV\",\"type\":\"foundation.two_phase_fluid.two_phase_fluid\"},{\"id\":\"AL\",\"label\":\"AL\",\"type\":\"foundation.two_phase_fluid.two_phase_fluid\"},{\"id\":\"H\",\"label\":\"H\",\"type\":\"foundation.thermal.thermal\"}],\"Right\":[{\"id\":\"BV\",\"label\":\"BV\",\"type\":\"foundation.two_phase_fluid.two_phase_fluid\"},{\"id\":\"BL\",\"label\":\"BL\",\"type\":\"foundation.two_phase_fluid.two_phase_fluid\"},{\"id\":\"L\",\"label\":\"L\",\"type\":\"output\"}],\"Top\":[]}"
  Reservoir (G) : fl_lib/Gas/Elements/Reservoir (G)  pressure_spec=foundation.enum.pressure_spec.atmospheric  reservoir_pressure=0.101325 MPa  reservoir_temperature=700 K  area_A=0.01 m^2
  Reservoir (TL)1 : fl_lib/Thermal Liquid/Elements/Reservoir (TL)  pressure_spec=foundation.enum.pressure_spec.atmospheric  reservoir_pressure=0.1 MPa  reservoir_temperature=293 K  area=0.01 m^2
  Reservoir (TL)2 : fl_lib/Thermal Liquid/Elements/Reservoir (TL)  pressure_spec=foundation.enum.pressure_spec.atmospheric  reservoir_pressure=0.1 MPa  reservoir_temperature=293 K  area=0.01 m^2
  Rotational Electromechanical Converter : fl_lib/Electrical/Electrical Elements/Rotational Electromechanical Converter  K=0.1 V*s/rad  i_specify=on  i_priority=None  i=0 A  i_nominal_specify=off  i_nominal_value=1  i_nominal_unit=A  v_specify=on  v_priority=None  v=0 V  v_nominal_specify=off  v_nominal_value=1  v_nominal_unit=V  t_specify=off  t_priority=None  t=0 N*m  t_nominal_specify=off  t_nominal_value=1  t_nominal_unit=N*m  w_specify=on  w_priority=None  w=314 rad/s  w_nominal_specify=off  w_nominal_value=1  w_nominal_unit=rad/s
  Rotational Inertia : fl_lib/Mechanical/Rotational Elements/Inertia  inertia=10 kg*m^2  num_ports=foundation.enum.numPorts2.one  w_specify=off  w_priority=High  w=0 rad/s  w_nominal_specify=off  w_nominal_value=1  w_nominal_unit=rad/s  t_specify=off  t_priority=None  t=0 N*m  t_nominal_specify=off  t_nominal_value=1  t_nominal_unit=N*m
  S-PS bypass : nesl_utility/Simulink-PS Converter  PhysicalDomain=network_engine_domain  SubClassName=ps_input  LeftPortType=input  RightPortType=output  PseudoPeriodic=off  Frequencies=[]  NoiseDistribution=none  NoiseParameters=[]  Unit=1  AffineConversion=off  FilteringAndDerivatives=provide  SimscapeFilterOrder=1  InputFilterTimeConstant=0.001  UdotUserProvided=0
  S-PS gas : nesl_utility/Simulink-PS Converter  PhysicalDomain=network_engine_domain  SubClassName=ps_input  LeftPortType=input  RightPortType=output  PseudoPeriodic=off  Frequencies=[]  NoiseDistribution=none  NoiseParameters=[]  Unit=1  AffineConversion=off  FilteringAndDerivatives=provide  SimscapeFilterOrder=1  InputFilterTimeConstant=0.001  UdotUserProvided=0
  S-PS nozzle : nesl_utility/Simulink-PS Converter  PhysicalDomain=network_engine_domain  SubClassName=ps_input  LeftPortType=input  RightPortType=output  PseudoPeriodic=off  Frequencies=[]  NoiseDistribution=none  NoiseParameters=[]  Unit=1  AffineConversion=off  FilteringAndDerivatives=provide  SimscapeFilterOrder=1  InputFilterTimeConstant=0.001  UdotUserProvided=0
  Scope : Scope
      settings: ActiveDisplayYMinimum=-20.986284031779046  ActiveDisplayYMaximum=188.83950834183415
  Simulink-PS Converter : nesl_utility/Simulink-PS Converter  PhysicalDomain=network_engine_domain  SubClassName=ps_input  LeftPortType=input  RightPortType=output  PseudoPeriodic=off  Frequencies=[]  NoiseDistribution=none  NoiseParameters=[]  Unit=1  AffineConversion=off  FilteringAndDerivatives=provide  SimscapeFilterOrder=1  InputFilterTimeConstant=0.001  UdotUserProvided=0
  Solver Configuration : nesl_utility/Solver Configuration  PhysicalDomain=network_engine_domain  SubClassName=solver  LeftPortType=input  RightPortType=generic  Tones=[]  Harmonics=[]  SimulateNoise=off  Profile=off  UseLocalSampling=off  EnableSwitchedLinearOptims=on  FrequencyDomain=off  UseCCode=off  RelTol=0.001  AbsTol=0.001  MinStep=1e-09  ToWorkspace=off  RevertToSquareIcSolve=off  NumHomotopyIterations=100  PhasorMode=off  PhasorModeNumHarmonics=1  ConsistencySolver=NEWTON_XTOL_AFTER_FTOL  IndexReductionMethod=DerivativeReplacement  DoDC=off  ResidualTolerance=1e-09  ConsistencyTolSource=GLOBAL  ConsistencyAbsTol=0.001  ConsistencyRelTol=0.001  ConsistencyTolFactor=0.001  UseLocalSolver=off  LocalSolverChoice=NE_BACKWARD_EULER_ADVANCER  ResolveIndetEquations=on  FunctionEvalNumThread=1  LocalSolverSampleTime=0.001  DoFixedCost=off  MaxNonlinIter=3  MaxModeIter=2  ComputeImpulses=off  ImpulseIterations=2  LinearAlgebra=auto  LinearAlgebraNumThread=0  EquationFormulation=NE_TIME_EF  DelaysMemoryBudget=1024  AutomaticFiltering=on  FilteringTimeConstant=0.001  PartitionStorageMethod=AS_NEEDED  PartitionMemoryBudget=1024  PartitionMethod=ROBUST  MultibodyUseLocalSolver=off  MultibodyLocalSolverChoice=ODE1  MultibodyLocalSolverSampleTime=0.001
  Solver Configuration1 : nesl_utility/Solver Configuration  PhysicalDomain=network_engine_domain  SubClassName=solver  LeftPortType=input  RightPortType=generic  Tones=[]  Harmonics=[]  SimulateNoise=off  Profile=off  UseLocalSampling=off  EnableSwitchedLinearOptims=on  FrequencyDomain=off  UseCCode=off  RelTol=0.001  AbsTol=0.001  MinStep=1e-09  ToWorkspace=off  RevertToSquareIcSolve=off  NumHomotopyIterations=100  PhasorMode=off  PhasorModeNumHarmonics=1  ConsistencySolver=NEWTON_XTOL_AFTER_FTOL  IndexReductionMethod=DerivativeReplacement  DoDC=off  ResidualTolerance=1e-09  ConsistencyTolSource=GLOBAL  ConsistencyAbsTol=0.001  ConsistencyRelTol=0.001  ConsistencyTolFactor=0.001  UseLocalSolver=off  LocalSolverChoice=NE_BACKWARD_EULER_ADVANCER  ResolveIndetEquations=on  FunctionEvalNumThread=1  LocalSolverSampleTime=0.001  DoFixedCost=off  MaxNonlinIter=3  MaxModeIter=2  ComputeImpulses=off  ImpulseIterations=2  LinearAlgebra=auto  LinearAlgebraNumThread=0  EquationFormulation=NE_TIME_EF  DelaysMemoryBudget=1024  AutomaticFiltering=on  FilteringTimeConstant=0.001  PartitionStorageMethod=AS_NEEDED  PartitionMemoryBudget=1024  PartitionMethod=ROBUST  MultibodyUseLocalSolver=off  MultibodyLocalSolverChoice=ODE1  MultibodyLocalSolverSampleTime=0.001
  Subsystem : Subsystem
  Subsystem1 : Subsystem
  Subsystem2 : Subsystem
  Subsystem3 : Subsystem
  Subsystem4 : Subsystem
  Subsystem5 : Subsystem
  Sum : Sum  Inputs=|+-
  Sum3 : Sum  Inputs=|+-
  Switch : Switch  Criteria=u2 > Threshold  Threshold=1  SaturateOnIntegerOverflow=off  InputSameDT=off
  T3_set : Constant  Value=ORC_T3set
  T_max : Constant  Value=GAS_Tmax
  Thermal Liquid Properties (TL)1 : SimscapeFluids_lib/Thermal Liquid/Utilities/Thermal Liquid Properties (TL)  fluid_list=fluids.thermal_liquid.utilities.enum.thermal_liquid_fluid_list.water  concentration_param_EG=fluids.thermal_liquid.utilities.enum.thermal_liquid_concentration.volume_fraction  concentration_param_PG=fluids.thermal_liquid.utilities.enum.thermal_liquid_concentration.volume_fraction  c_mass_SW=3.5e-3  c_mass_EG=0.1  c_mass_PG=0.1  c_mass_GL=0.1  c_vol_EG=0.1  c_vol_PG=0.1  beta_const_EG=2.1791 GPa  beta_const_PG=2.1791 GPa  beta_const_GL=2.1791 GPa  p_min_EG=0.01 MPa  p_min_PG=0.01 MPa  p_min_GL=0.01 MPa  p_max_EG=50 MPa  p_max_PG=50 MPa  p_max_GL=50 MPa  p_atm=0.101325 MPa  properties_range_check=simscape.enum.assert.action.error
  Torquee : nesl_utility/Simulink-PS Converter  PhysicalDomain=network_engine_domain  SubClassName=ps_input  LeftPortType=input  RightPortType=output  PseudoPeriodic=off  Frequencies=[]  NoiseDistribution=none  NoiseParameters=[]  Unit=1  AffineConversion=off  FilteringAndDerivatives=filter  SimscapeFilterOrder=1  InputFilterTimeConstant=0.001  UdotUserProvided=0
  Turbine (2P) : SimscapeFluids_lib/Two-Phase Fluid/Fluid Machines/Turbine (2P)  parameterization=fluids.two_phase_fluid.fluid_machines.enum.TurbineParameterization.Analytical  omega_TLU_2=[12500, 15000, 17500, 20000, 22500, 25000, 27500] rpm  variable_nozzle=true  min_nozzle_opening=1e-3  max_nozzle_opening=1.  pr_nom=TRB_pr  mdot_nom=TRB_mdot kg/s  pr_mdot_TLU=[1.251, 1.345, 1.442, 1.521, 1.596, 1.692, 1.849, 1.972, 2.1, 2.173, 2.259, 2.3424]  mdot_TLU=0.01 .* [39.439, 43.01, 45.556, 46.801, 47.792, 48.388, 48.634, 48.67, 48.689, 48.747, 48.825, 48.912] kg/s  pr_mdot_TLU_2=[1.217, 1.285, 1.323, 1.363, 1.402, 1.427, 1.495, 1.545, 1.6, 1.687, 1.747, 1.8074; 1.231, 1.302, 1.356, 1.404, 1.443, 1.473, 1.525, 1.577, 1.635, 1.709, 1.782, 1.845; 1.242, 1.328, 1.388, 1.437, 1.528, 1.617, 1.704, 1.811, 1.915, 1.979, 2.053, 2.1226; 1.244, 1.339, 1.417, 1.465, 1.528, 1.584, 1.692, 1.787, 1.899, 2, 2.075, 2.1492; 1.245, 1.34, 1.425, 1.492, 1.546, 1.684, 1.748, 1.882, 1.987, 2.084, 2.167, 2.2458; 1.251, 1.345, 1.442, 1.521, 1.596, 1.692, 1.849, 1.972, 2.1, 2.173, 2.259, 2.3424; 1.248, 1.348, 1.447, 1.516, 1.581, 1.651, 1.749, 1.839, 1.93, 2.024, 2.154, 2.242]  mdot_TLU_2=0.01 .* [40.403, 44.417, 46.653, 47.966, 48.97, 49.544, 50.001, 50.081, 50.086, 50.095, 50.09, 50.0922; 40.044, 43.754, 46.125, 47.626, 48.513, 49.105, 49.481, 49.58, 49.597, 49.624, 49.638, 49.633; 39.941, 43.795, 46.017, 47.335, 48.795, 49.199, 49.279, 49.27, 49.248, 49.23, 49.255, 49.2428; 39.896, 43.512, 45.914, 47.061, 48.011, 48.558, 48.943, 49.042, 49.069, 49.01, 49.046, 49.0266; 39.524, 42.934, 45.686, 46.743, 47.715, 48.67, 48.777, 48.836, 48.876, 48.836, 48.845, 48.8184; 39.439, 43.01, 45.556, 46.801, 47.792, 48.388, 48.634, 48.67, 48.639, 48.647, 48.625, 48.5912; 39.502, 42.849, 45.336, 46.385, 47.312, 47.877, 48.222, 48.397, 48.459, 48.482, 48.455, 48.414] kg/s  efficiency_constant=0.8  pr_eta_TLU=[1.252, 1.328, 1.425, 1.544, 1.642, 1.757, 1.873, 2.005, 2.1, 2.204, 2.248, 2.28]  eta_TLU=[.559, .61, .673, .741, .788, .835, .869, .895, .908, .899, .854, .751]  pr_eta_TLU_2=[1.224, 1.246, 1.292, 1.387, 1.457, 1.534, 1.61, 1.686, 1.743, 1.79, 1.871, 1.914; 1.237, 1.25, 1.28, 1.369, 1.459, 1.553, 1.629, 1.716, 1.799, 1.846, 1.927, 1.97; 1.241, 1.255, 1.283, 1.326, 1.401, 1.509, 1.591, 1.704, 1.806, 1.913, 1.994, 2.037; 1.25, 1.265, 1.308, 1.364, 1.456, 1.532, 1.637, 1.739, 1.851, 1.934, 2.042, 2.085; 1.281, 1.314, 1.371, 1.425, 1.498, 1.574, 1.647, 1.749, 1.878, 1.979, 2.091, 2.18; 1.252, 1.328, 1.425, 1.544, 1.642, 1.757, 1.873, 2.005, 2.1, 2.204, 2.248, 2.28; 1.382, 1.43, 1.495, 1.586, 1.688, 1.791, 1.887, 1.99, 2.079, 2.158, 2.249, 2.36]  eta_TLU_2=[.72, .754, .759, .739, .714, .679, .643, .603, .554, .524, .494, .48; .716, .757, .794, .819, .812, .788, .761, .728, .692, .662, .632, .618; .629, .691, .775, .831, .858, .869, .859, .842, .816, .782, .752, .738; .594, .668, .757, .804, .857, .883, .892, .893, .884, .865, .835, .821; .664, .72, .779, .823, .858, .883, .897, .905, .904, .896, .883, .868; .559, .61, .673, .741, .788, .835, .869, .895, .908, .899, .854, .751; .718, .785, .824, .855, .882, .9, .908, .906, .884, .857, .804, .701]  p_reference=ORC_pset_MPa MPa  T_reference=TRB_Tref K  mechanical_efficiency=0.9  area_A=0.01 m^2  area_B=0.01 m^2  vapor_check=simscape.enum.assert.action.warn
      settings: InternalSimscapePortConfiguration="{\"Bottom\":[],\"Left\":[{\"id\":\"A\",\"label\":\"A\",\"type\":\"foundation.two_phase_fluid.two_phase_fluid\"},{\"id\":\"R\",\"label\":\"R\",\"type\":\"foundation.mechanical.rotational.rotational\"},{\"id\":\"VN\",\"label\":\"VN\",\"type\":\"input\"}],\"Right\":[{\"id\":\"B\",\"label\":\"B\",\"type\":\"foundation.two_phase_fluid.two_phase_fluid\"},{\"id\":\"C\",\"label\":\"C\",\"type\":\"foundation.mechanical.rotational.rotational\"}],\"Top\":[]}"
  Two-Phase Fluid Predefined Properties (2P) : SimscapeFluids_lib/Two-Phase Fluid/Utilities/Two-Phase Fluid Predefined Properties (2P)  fluid=fluids.two_phase_fluid.utilities.enum.Fluid.R1233zdE  p_atm=0.101325 MPa  properties_range_check=simscape.enum.assert.action.error  q_rev=0.01 Pa
  e_T3 : Sum  Inputs=-+
  e_Tmax : Sum  Inputs=-+
  e_p : Sum  Inputs=-+
  gas bypass : Sum  Inputs=+-
  gas cmd : Saturate  UpperLimit=GAS_total  LowerLimit=GAS_min  ZeroCross=off
  gas guard : Product
  gas to HRS : MinMax  Inputs=2
  k_Tmax : Gain  Gain=1/GAS_dT
  log_ORC_mexh : ToWorkspace  VariableName=ORC_mexh  SaveFormat=Timeseries  SampleTime=-1
  log_ORC_mgas : ToWorkspace  VariableName=ORC_mgas  SaveFormat=Timeseries  SampleTime=-1
  log_ORC_mwf : ToWorkspace  VariableName=ORC_mwf  SaveFormat=Timeseries  SampleTime=-1
  log_ORC_noz : ToWorkspace  VariableName=ORC_noz  SaveFormat=Timeseries  SampleTime=-1
  log_ORC_w : ToWorkspace  VariableName=ORC_w  SaveFormat=Timeseries  SampleTime=-1
  m_dot : Constant  Value=NOZ_u0
  p_set : Constant  Value=ORC_pset_MPa*1e6
  sat_Tmax : Saturate  UpperLimit=1  LowerLimit=0  ZeroCross=off
  EVAP : PMIOPort  Side=Right
  - : PMIOPort  Port=2  Side=Right
  + : PMIOPort  Port=3  Side=Right
  IGEN : Outport
  Out1 : Outport  Port=2
  wires:
  PS-Simulink Converter22/1 -> Scope/1, IGEN/1
  PS-Simulink Converter12/1 -> Sum3/1
  In1/1 -> Sum3/2
  Sum3/1 -> PID Controller2/1
  PID Controller2/1 -> Out1/1
  Omega1/1 -> [Omega], log_ORC_w/1
  Constant2/1 -> Load Torque/3(In3)
  Load Torque/1(Out1) -> Torquee/1
  Clock/1 -> Load Torque/2(In2)
  Constant1/1 -> Load Torque/1(In1)
  [m_dot_2] -> Switch/1
  Clock1/1 -> Switch/2
  m_dot/1 -> Switch/3
  Sum/1 -> PID Controller/1
  PID Controller/1 -> [m_dot_2]
  [Omega] -> Sum/2
  Constant3/1 -> Sum/1
  Switch/1 -> S-PS nozzle/1, log_ORC_noz/1
  [ORC_P3] -> e_p/1
  p_set/1 -> e_p/2
  e_p/1 -> PI pump/1
  PI pump/1 -> log_ORC_mwf/1, Simulink-PS Converter/1
  [ORC_T3] -> e_T3/1
  T3_set/1 -> e_T3/2
  e_T3/1 -> PI gas/1
  [ORC_T3] -> e_Tmax/1
  T_max/1 -> e_Tmax/2
  e_Tmax/1 -> k_Tmax/1
  k_Tmax/1 -> sat_Tmax/1
  PI gas/1 -> gas guard/1
  sat_Tmax/1 -> gas guard/2
  gas guard/1 -> gas cmd/1
  gas cmd/1 -> gas to HRS/1
  Exhaust available/1 -> gas bypass/1, gas to HRS/2, log_ORC_mexh/1
  gas to HRS/1 -> S-PS gas/1, log_ORC_mgas/1, gas bypass/2
  gas bypass/1 -> S-PS bypass/1
  connections:
  PS-Simulink Converter22/LConn1 -- Current Sensor/RConn1
  Flow Rate Source (G)/LConn1 -- Bypass (G)/LConn1 -- Subsystem4/LConn1 -- Reservoir (G)/LConn1 -- Gas Properties (G)/RConn1
  Rotational Electromechanical Converter/LConn1 -- Current Sensor/LConn1
  Rotational Inertia/LConn1 -- Turbine (2P)/LConn2 -- Rotational Electromechanical Converter/LConn2 -- Ideal Torque Source/LConn1 -- Ideal Rotational Motion Sensor1/LConn1
  Two-Phase Fluid Predefined Properties (2P)/RConn1 -- Solver Configuration/RConn1 -- Subsystem1/LConn1 -- Subsystem1/LConn2 -- Pump/LConn1 -- Receiver (2P)/RConn2
  Mechanical Rotational Reference5/LConn1 -- Rotational Electromechanical Converter/RConn2
  Condenser Evaporator (TL-2P)1/RConn1 -- Turbine (2P)/RConn1 -- Subsystem/LConn2 -- Subsystem/LConn1
  Turbine (2P)/LConn1 -- Subsystem3/LConn2 -- Subsystem3/LConn1 -- Condenser Evaporator (2P-G)/LConn2
  Condenser Evaporator (2P-G)/LConn1 -- Subsystem2/LConn2 -- Subsystem2/LConn1 -- Pump/RConn1
  Flow Rate Source (TL)1/RConn1 -- Condenser Evaporator (TL-2P)1/LConn1
  Electrical Reference1/LConn1 -- Rotational Electromechanical Converter/RConn1 -- -/RConn1
  Turbine (2P)/RConn2 -- Mechanical Rotational Reference/LConn1
  Reservoir (TL)1/LConn1 -- Thermal Liquid Properties (TL)1/RConn1 -- Flow Rate Source (TL)1/LConn1
  Reservoir (TL)2/LConn1 -- Condenser Evaporator (TL-2P)1/LConn2
  Flow Rate Source (G)/RConn1 -- Subsystem5/LConn1 -- Condenser Evaporator (2P-G)/RConn1
  EVAP/RConn1 -- Condenser Evaporator (2P-G)/RConn2 -- Bypass (G)/RConn1
  +/RConn1 -- Current Sensor/RConn2
  PS-Simulink Converter12/LConn1 -- PS Constant/RConn1 -- Solver Configuration1/RConn1
  Torquee/RConn1 -- Ideal Torque Source/RConn1
  Omega1/LConn1 -- Ideal Rotational Motion Sensor1/RConn2
  Mechanical Rotational Reference1/LConn1 -- Ideal Torque Source/RConn2
  Mechanical Rotational Reference3/LConn1 -- Ideal Rotational Motion Sensor1/RConn1
  Simulink-PS Converter/RConn1 -- Pump/LConn2
  Condenser Evaporator (TL-2P)1/RConn2 -- Receiver (2P)/LConn2
  S-PS nozzle/RConn1 -- Turbine (2P)/LConn3
  S-PS gas/RConn1 -- Flow Rate Source (G)/LConn2
  S-PS bypass/RConn1 -- Bypass (G)/LConn2
